simulink model "turbo_controller"  (R2025a)
settings: Solver=FixedStepAuto  StartTime=0.0  StopTime=inf  FixedStep=0.001  RelTol=1e-3
PostLoadFcn:
  | % 自动定位同目录CubeMX文件；不需要外部初始化脚本。
  | codertarget.data.setParameterValue('turbo_controller','STM32CubeMX.ProjectFile',fullfile(fileparts(get_param('turbo_controller','FileName')),'turbo_f407.ioc'));
InitFcn:
  | % 中文说明：按原控制器字段与类型创建三组接口总线；控制参数已内嵌。
  | tc_names=["EValve_Cycle" "EValve_Open" "Eblast_Cycle" "Eblast_Open" "Motor_Cycle" "Motor_Open" "EValve_Enable" "Eblast_Enable" "Motor_Enable" "SWO_Firework" "SWO_BleedAir" "EngineState" "Flag_ECUReset_Clear" "Flag_ECUReset_Save" "Flag_Reset_Enable" "Accelerator" "Nc_dem" "Nc"]; tc_types=["uint16" "uint16" "uint16" "uint16" "uint16" "uint16" "uint8" "uint8" "uint8" "uint8" "uint8" "uint8" "uint8" "uint8" "uint8" "single" "single" "single"];
  | for tc_k=1:numel(tc_names)
  |  tc_e(tc_k)=Simulink.BusElement; tc_e(tc_k).Name=char(tc_names(tc_k)); tc_e(tc_k).DataType=char(tc_types(tc_k));
  | end
  | EngineControl_Out=Simulink.Bus; EngineControl_Out.DataScope='Exported'; EngineControl_Out.Elements=tc_e;
  | clear tc_e tc_names tc_types tc_k
  | tc_names=["savedata1" "savedata2" "savedata3" "savedata4" "savedata5" "savedata6" "savedata7" "savedata8" "savedata9" "savedata10" "savedata11" "savedata12" "savedata13" "savedata14" "savedata15" "savedata16" "savedata17" "savedata18" "savedata19" "savedata20" "savedata21" "savedata22" "savedata23" "savedata24" "savedata25"]; tc_types=["single" "single" "single" "single" "single" "single" "single" "single" "single" "single" "single" "single" "single" "single" "single" "single" "single" "single" "single" "single" "single" "single" "single" "single" "single"];
  | for tc_k=1:numel(tc_names)
  |  tc_e(tc_k)=Simulink.BusElement; tc_e(tc_k).Name=char(tc_names(tc_k)); tc_e(tc_k).DataType=char(tc_types(tc_k));
  | end
  | SaveData_Out=Simulink.Bus; SaveData_Out.DataScope='Exported'; SaveData_Out.Elements=tc_e;
  | clear tc_e tc_names tc_types tc_k
  | tc_names=["senddata1" "senddata2" "senddata3" "senddata4" "senddata5" "senddata6" "senddata7" "senddata8" "senddata9" "senddata10" "senddata11" "senddata12" "senddata13" "senddata14" "senddata15" "senddata16" "senddata17" "senddata18" "senddata19" "senddata20" "senddata21" "senddata22" "senddata23" "senddata24" "senddata25" "senddata26" "senddata27" "senddata28" "senddata29"]; tc_types=["uint8" "uint8" "uint8" "uint8" "uint8" "uint8" "uint8" "uint8" "uint8" "uint8" "uint8" "uint8" "uint8" "uint8" "uint8" "uint8" "uint8" "uint8" "uint8" "uint8" "uint8" "uint8" "uint8" "uint8" "uint8" "uint8" "uint8" "uint8" "uint8"];
  | for tc_k=1:numel(tc_names)
  |  tc_e(tc_k)=Simulink.BusElement; tc_e(tc_k).Name=char(tc_names(tc_k)); tc_e(tc_k).DataType=char(tc_types(tc_k));
  | end
  | SendData_Out=Simulink.Bus; SendData_Out.DataScope='Exported'; SendData_Out.Elements=tc_e;
  | clear tc_e tc_names tc_types tc_k
  | 
  | % 以下为接口中文说明；只设置描述，不改变数值或数据类型。
  | EngineControl_Out.Description='执行控制输出（阀、电机、点火、状态及复位请求）';
  | tc_cn=["EValve_Cycle（主油阀周期计数（每计数2毫秒））" "EValve_Open（主油阀开通计数（每计数2毫秒））" "Eblast_Cycle（副油阀周期计数（每计数2毫秒））" "Eblast_Open（副油阀开通计数（每计数2毫秒））" "Motor_Cycle（起动电机周期计数）" "Motor_Open（起动电机开通计数）" "EValve_Enable（主油阀驱动使能）" "Eblast_Enable（副油阀驱动使能）" "Motor_Enable（起动电机使能）" "SWO_Firework（点火器使能（1开））" "SWO_BleedAir（引气阀使能（1开））" "EngineState（发动机状态）" "Flag_ECUReset_Clear（清除复位恢复状态请求）" "Flag_ECUReset_Save（保存复位恢复数据请求）" "Flag_Reset_Enable（处理器软件复位请求）" "Accelerator（油门／油泵给定控制量）" "Nc_dem（控制目标转速）" "Nc（发动机反馈转速（转每分））"];
  | tc_elements=EngineControl_Out.Elements;
  | for tc_k=1:numel(tc_cn)
  |  tc_elements(tc_k).Description=char(tc_cn(tc_k));
  | end
  | EngineControl_Out.Elements=tc_elements;
  | clear tc_cn tc_elements tc_k
  | SaveData_Out.Description='25项运行记录；字段含义按当前模型数据来源解释';
  | tc_cn=["savedata1（指令回显记录）" "savedata2（入口总温记录（℃））" "savedata3（电源电压记录）" "savedata4（排气温度记录（℃））" "savedata5（标定燃油压力记录）" "savedata6（副油阀占空比记录（％））" "savedata7（主油阀占空比记录（％））" "savedata8（温度修正转速记录）" "savedata9（开关输出及反馈位域）" "savedata10（物理转速记录）" "savedata11（油泵目标给定原始值）" "savedata12（起动电机占空比记录（％））" "savedata13（发动机状态码记录）" "savedata14（故障告警位域记录）" "savedata15（模型记录帧序号）" "savedata16（处理器温度记录（℃））" "savedata17（装订转速记录（沿用旧电源字段名））" "savedata18（导航高度记录）" "savedata19（飞行空速记录）" "savedata20（主阀旧记录位（恒零保留））" "savedata21（第21项保留记录（恒零））" "savedata22（保留记录项22）" "savedata23（保留记录项23）" "savedata24（保留记录项24）" "savedata25（保留记录项25）"];
  | tc_elements=SaveData_Out.Elements;
  | for tc_k=1:numel(tc_cn)
  |  tc_elements(tc_k).Description=char(tc_cn(tc_k));
  | end
  | SaveData_Out.Elements=tc_elements;
  | clear tc_cn tc_elements tc_k
  | SendData_Out.Description='29字段回传及外设命令接口；板端上位机帧只取第3至27字段';
  | tc_cn=["senddata1（回传发送允许标志（不直接上线路））" "senddata2（回传载荷长度25字节）" "senddata3（回传指令回显字节）" "senddata4（总温编码字节（℃＋80））" "senddata5（电源电压编码字节）" "senddata6（排温编码高字节）" "senddata7（排温编码低字节）" "senddata8（燃油压力编码高字节）" "senddata9（燃油压力编码低字节）" "senddata10（副油阀占空比字节（％））" "senddata11（主油阀占空比字节（％））" "senddata12（修正转速编码高字节）" "senddata13（修正转速编码低字节）" "senddata14（驱动及反馈状态位域）" "senddata15（物理转速编码高字节）" "senddata16（物理转速编码低字节）" "senddata17（油泵目标给定高字节（串口二使用））" "senddata18（油泵目标给定低字节（串口二使用））" "senddata19（起动电机占空比命令（串口一使用））" "senddata20（发动机状态码字节）" "senddata21（故障告警位域字节）" "senddata22（帧序号占位（板端另行填写））" "senddata23（处理器温度编码（℃＋50））" "senddata24（控制目标转速编码高字节）" "senddata25（控制目标转速编码低字节）" "senddata26（占位字节（板端改填实测泵速高字节））" "senddata27（占位字节（板端改填实测泵速低字节））" "senddata28（装订转速高字节（本板未发送））" "senddata29（装订转速低字节（本板未发送））"];
  | tc_elements=SendData_Out.Elements;
  | for tc_k=1:numel(tc_cn)
  |  tc_elements(tc_k).Description=char(tc_cn(tc_k));
  | end
  | SendData_Out.Elements=tc_elements;
  | clear tc_cn tc_elements tc_k
  | 
  | 
  | % FRAM模块化事务：接口类型和上电初始状态，随模型保存，无外部初始化文件。
  | clear FM_elements
  | FM_elements(1)=Simulink.BusElement;FM_elements(1).Name='phase';FM_elements(1).DataType='uint8';FM_elements(1).Dimensions=[1 1];FM_elements(1).Description='phase（当前事务阶段）';
  | FM_elements(2)=Simulink.BusElement;FM_elements(2).Name='a';FM_elements(2).DataType='uint8';FM_elements(2).Dimensions=[64 1];FM_elements(2).Description='a（启动时缓存的首区64字节）';
  | FM_elements(3)=Simulink.BusElement;FM_elements(3).Name='active';FM_elements(3).DataType='uint16';FM_elements(3).Dimensions=[1 1];FM_elements(3).Description='active（当前有效记录区地址）';
  | FM_elements(4)=Simulink.BusElement;FM_elements(4).Name='generation';FM_elements(4).DataType='uint32';FM_elements(4).Dimensions=[1 1];FM_elements(4).Description='generation（当前有效记录代号）';
  | FM_elements(5)=Simulink.BusElement;FM_elements(5).Name='record';FM_elements(5).DataType='uint8';FM_elements(5).Dimensions=[64 1];FM_elements(5).Description='record（本次冻结的待写记录）';
  | FM_elements(6)=Simulink.BusElement;FM_elements(6).Name='addr';FM_elements(6).DataType='uint16';FM_elements(6).Dimensions=[1 1];FM_elements(6).Description='addr（本次备用写入地址）';
  | FM_elements(7)=Simulink.BusElement;FM_elements(7).Name='lastSave';FM_elements(7).DataType='single';FM_elements(7).Dimensions=[1 1];FM_elements(7).Description='lastSave（上次开始保存的秒数）';
  | FM_elements(8)=Simulink.BusElement;FM_elements(8).Name='lastState';FM_elements(8).DataType='uint8';FM_elements(8).Dimensions=[1 1];FM_elements(8).Description='lastState（上次保存时的发动机状态）';
  | FM_elements(9)=Simulink.BusElement;FM_elements(9).Name='boot';FM_elements(9).DataType='boolean';FM_elements(9).Dimensions=[1 1];FM_elements(9).Description='boot（启动记录是否允许恢复）';
  | FM_elements(10)=Simulink.BusElement;FM_elements(10).Name='consumed';FM_elements(10).DataType='boolean';FM_elements(10).Dimensions=[1 1];FM_elements(10).Description='consumed（本次启动恢复通知是否已发送）';
  | FM_elements(11)=Simulink.BusElement;FM_elements(11).Name='payload';FM_elements(11).DataType='uint8';FM_elements(11).Dimensions=[20 1];FM_elements(11).Description='payload（当前20字节恢复内容）';
  | ... (+35 lines)
model workspace (MAT data in the model file):
  CRC16_Table_Reference = [0 4129 8258 12387 16516 20645 24774 28903 33032 37161 41290 45419 ... (256 elements, 256x1)]
  PE_Kaer = [0.15402 0.15402 0.12264 0.10076 0.09481 0.07601 0.07111 0.0569 0.05198 0.04926 0.05308 0.04325 ... (13 elements, 1x13)]
  PE_Nr = [21.2982 61.4260372 67.7475458 72.7394382 76.845934 80.6988798 83.8449282 86.6491912 88.9382406 89.178606 91.1938214 93.4068058 ... (13 elements, 1x13)]
  PE_Pump_Translate = 33.5999984741
  PE_RotaSpeed_Translate = 860
  PE_Taer = [0.4939154 0.4939154 0.40780982 0.34066978 0.31622756 0.30405716 0.34300244 0.26785022 0.37393554 0.23914836 0.44563948 0.31044662 ... (13 elements, 1x13)]
  PF_ACCFULLRANGE = 3360
  PF_Flag_ECUReset = 0
  PF_Flag_rx_suc = 1
  PF_Gear_Info = [40000; 45000; 50000; 55000; 57000; 59000; 60000; 61000; 61000; 61000; 61000; 61000]
  PF_K_TiaoJie = 1
  PF_Kpu = 10
  PF_MySet_Rxdata = [0 0 0 0 0 0 0 0 0 0 0 0 ... (50 elements, 50x1)]
  PF_MyUsart1_Rxdata = [0 0 0 0 0 0 0 0 0 0 0 0 ... (50 elements, 50x1)]
  PF_MyUsart2_Rxdata = [0 0 0 0 0 0 0 0 0 0 0 0 ... (50 elements, 50x1)]
  PF_Reset_Information = [0 0 0 0 0 0 0 0 0 0 0 0 ... (20 elements, 20x1)]
  PF_Sensor_X1_T4 = [0 4095]
  PF_Sensor_X2_T4 = [0 1.66666698456]
  PF_Sensor_X3_T4 = [0 504 999 1497 2010 2529 3051 3568 4076 4571 4959]
  PF_Sensor_X_P2 = [0.5 3]
  PF_Sensor_X_Poil = [0.5 3]
  PF_Sensor_X_T1t = [-50 300]
  PF_Sensor_X_Vpower = [0 3]
  PF_Sensor_X_Vpump = [0 3]
  PF_Sensor_Y1_T4 = [0 3]
  PF_Sensor_Y2_T4 = [0 5000]
  PF_Sensor_Y3_T4 = [0 100 200 300 400 500 600 700 800 900 980]
  PF_Sensor_Y_P2 = [0 1000]
  PF_Sensor_Y_Poil = [0 1000]
  PF_Sensor_Y_T1t = [-50 300]
  PF_Sensor_Y_Vpower = [0 33]
  PF_Sensor_Y_Vpump = [0 33]
  PG_CtrlMode_CloseLoop : mpt.Parameter (value not decoded)
  PG_CtrlMode_ManualAcc : mpt.Parameter (value not decoded)
  PG_CtrlMode_Origin : mpt.Parameter (value not decoded)
  PG_CtrlMode_Start : mpt.Parameter (value not decoded)
  PG_CtrlMode_Stop : mpt.Parameter (value not decoded)
  PG_ES_Clp : mpt.Parameter (value not decoded)
  PG_ES_EngStart : mpt.Parameter (value not decoded)
  PG_ES_Manual : mpt.Parameter (value not decoded)
  PG_ES_Origin : mpt.Parameter (value not decoded)
  PG_ES_Stop : mpt.Parameter (value not decoded)
  PG_Instr_BleedAirSet : mpt.Parameter (value not decoded)
  PG_Instr_CloseLoop : mpt.Parameter (value not decoded)
  PG_Instr_ECUReSet : mpt.Parameter (value not decoded)
  PG_Instr_EValveSet : mpt.Parameter (value not decoded)
  PG_Instr_EblastSet : mpt.Parameter (value not decoded)
  PG_Instr_Erase : mpt.Parameter (value not decoded)
  PG_Instr_FireWorkSet : mpt.Parameter (value not decoded)
  PG_Instr_ManualPlus : mpt.Parameter (value not decoded)
  PG_Instr_ManualrReduce : mpt.Parameter (value not decoded)
  PG_Instr_MotorSet : mpt.Parameter (value not decoded)
  PG_Instr_OilSet : mpt.Parameter (value not decoded)
  PG_Instr_SelfCheck : mpt.Parameter (value not decoded)
  PG_Instr_Start : mpt.Parameter (value not decoded)
  PG_Instr_Stop : mpt.Parameter (value not decoded)
  PG_Instr_StopZero : Simulink.Parameter (value not decoded)
  PG_Location_Air : Simulink.Parameter (value not decoded)
  PG_Location_Gnd : Simulink.Parameter (value not decoded)
  PG_ServoCtrlMode_CloseLoop : Simulink.Parameter (value not decoded)
  PG_ServoCtrlMode_CloseLoopMax : Simulink.Parameter (value not decoded)
  PG_ServoCtrlMode_CloseLoopMin : Simulink.Parameter (value not decoded)
  PG_ServoCtrlMode_ManualAcc : Simulink.Parameter (value not decoded)
  PG_ServoCtrlMode_ManualAccMax : Simulink.Parameter (value not decoded)
  PG_ServoCtrlMode_ManualAccMin : Simulink.Parameter (value not decoded)
  PG_SpeedDot_Permit : Simulink.Parameter (value not decoded)
  PL_EngineModel_Actuator = [0 10 100]
  PL_EngineModel_EngineStar_Press_P2 = [1013 1098.4 1099.144828 1099.931034 1103.613793 1162.662069 1143.793103 1131.006897 1123.186207 1117.6 1114 1111.806897 ... (127 elements, 1x127)]
  PL_EngineModel_EngineStar_RotaSpeed = [200 2000 9584 9660 10220 10240 10260 10288 10308 10368 10380 10408 ... (127 elements, 1x127)]
  PL_EngineModel_EngineStar_Temp_Exhaust = [128 129 129.1 130 131 131.1 132 133 134 134.1 135 135.1 ... (127 elements, 1x127)]
  PL_EngineModel_EngineStar_Time = [0.05 0.1 0.15 0.2 0.25 0.3 0.35 0.4 0.45 0.5 0.55 0.6 ... (127 elements, 1x127)]
  PL_EngineModel_IdleAbove_Nr = [0 21.2982 61.4260372 67.7475458 72.7394382 76.845934 80.6988798 83.8449282 86.6491912 88.9382406 89.178606 91.1938214 ... (14 elements, 1x14)]
  PL_EngineModel_IdleAbove_P2r = [0.986923266716 1.57907722675 1.81593881076 1.99358499877 2.23044658278 2.43770046879 2.65482358747 2.84233900814 3.03972366149 3.18776215149 3.25684678016 3.3950160375 ... (14 elements, 1x14)]
  PL_EngineModel_IdleAbove_Tempr = [0.0536001429337 1.07200285867 1.63301768805 1.63659103091 1.66875111667 1.72592460247 1.77595140254 1.86171163123 1.95461854565 2.03323208862 2.03323208862 2.13685903162 ... (14 elements, 1x14)]
  PL_EngineModel_IdleAbove_Ter = [0.42434128 0.42434128 0.42434128 0.30669408 0.23570008 0.22150128 0.1997974 0.23803274 0.16115638 0.24279948 0.13600422 0.31308354 ... (14 elements, 1x14)]
  PL_EngineModel_IdleAbove_Wfr = [0 10.142 23.8337 27.8905 31.9473 36.0041 40.0609 44.1177 48.1745 52.2313 52.7384 56.7952 ... (14 elements, 1x14)]
  PL_EngineModel_Press_P2 = [400 400 400 400 400 400 400 400 400 400]
  PL_EngineModel_Rotaspeed = [0 20000 96400]
  PL_EngineModel_Temp_Exhaust = [500 500 500 500 500 500 500 500 500 500]
  PL_Kaer = [0.1 0.1 0.1 0.1 0.1 0.1]
  PL_Nr = [50 60 70 80 90 100]
  PL_Taer = [0.1 0.1 0.1 0.1 0.1 0.1]
  Sig : Simulink.Signal (value not decoded)
  Ts_ms : Simulink.Parameter (value not decoded)
  false : Simulink.Parameter (value not decoded)
  true : Simulink.Parameter (value not decoded)
symbols that are objects in the model workspace (value not decoded): PG_CtrlMode_CloseLoop, PG_CtrlMode_ManualAcc, PG_CtrlMode_Origin, PG_CtrlMode_Start, PG_CtrlMode_Stop, PG_ES_Clp, PG_ES_EngStart, PG_ES_Manual, PG_ES_Origin, PG_ES_Stop, PG_Instr_BleedAirSet, PG_Instr_CloseLoop, PG_Instr_EblastSet, PG_Instr_ECUReSet, PG_Instr_Erase, PG_Instr_EValveSet, PG_Instr_FireWorkSet, PG_Instr_ManualPlus, PG_Instr_ManualrReduce, PG_Instr_MotorSet, PG_Instr_OilSet, PG_Instr_SelfCheck, PG_Instr_Start, PG_Instr_Stop, PG_Instr_StopZero, PG_ServoCtrlMode_CloseLoop, PG_ServoCtrlMode_CloseLoopMax, PG_ServoCtrlMode_CloseLoopMin, PG_ServoCtrlMode_ManualAcc, PG_ServoCtrlMode_ManualAccMax, PG_ServoCtrlMode_ManualAccMin, Ts_ms
libraries: simulink x97, stm32blockslib x10, stm32f4xxblockslib x8
(part 25 of 26)

== stateflow chart turbo_controller/CLM/Start/Start_OpenLoop ==
  note: 普通起动的六阶段顺序控制
      |
      | A准备：等待约1 s，记录并限制起动前油压参考，设置阀门周期、开启主副油路及电机使能。
      | B拖转：转速达到1000后进入C，开启点火并给出起动供油；约6 s仍未达到要求时走异常退出。
      | C建立油路：经过约3 s、油压相对基准上升50或已有进入标志时，调整主油阀与泵给定；按t、T参数和
      | 转速条件逐渐提高电机开通，达到100进入D。
      | D继续加速：转速超过参数n1进入E；超过约6 s未满足条件时撤销点火、清供油并设置异常阶段码。
      | E按转速供油：泵给定在(n1,m1)、(n2,m2)间按直线计算；超过13000时撤销起动电机和点火，超过2000
      | 0进入F。油压持续高于700或本阶段约30 s超时也有退出分支。
      | F转闭环：转速超过28000或达到约20 s时关闭副油路；再按1 s、3 s的延迟恢复主油路和m4给定，最后
      | 申请进入闭环。
      |
      | 转速单位rpm，T4为温度，油压阈值采用标定后的工程编码。计时统一按毫秒/Ts_ms比较；Ts_ms=20 ms
      | 时，1000 ms对应50次调用。泵曲线公式：
      | 泵给定=m1+(m2-m1)×(当前转速-n1)/(n2-n1)。
      |
      | 这些阶段是流程标志，不是额外的AirStart或BWStart模式。电机关闭还有高转速及锁存路径，最终输
      | 出仍受父级模式和使能控制。
  (default) -> (junction 24)
    settings: description=无附加条件的迁移路径，执行次序1；沿本图当前连接推进。
  (junction 24) -> (junction 458) [order 1] : [Start_A/*起动阶段或中间量编号*/  == true/*真值*/]
    settings: description=本路径的判据/动作：[Start_A == true]。执行次序1；条件成立才执行本箭头动作。
  (junction 458) -> (junction 1346) [order 1] : [CNT_Start_A/*计数器起动阶段或中间量编号*/ >= (1000/Ts_ms/*采样周期毫秒*/)]
    settings: description=本路径的判据/动作：[CNT_Start_A >= (1000/Ts_ms)]。执行次序1；条件成立才执行本箭头动作。
  (junction 1346) -> (junction 1355) [order 1] : [POil/*标定燃油压力*/<50]
    settings: description=本路径的判据/动作：[POil<50]。执行次序1；条件成立才执行本箭头动作。
  (junction 24) -> (junction 463) [order 2]
    settings: description=无附加条件的迁移路径，执行次序2；沿本图当前连接推进。
  (junction 458) -> (junction 466) [order 2] : {Motor_Cycle/*起动电机周期计数*/ = 100;
      | Motor_Open/*起动电机开通计数*/ = NPump0/*油泵转速0*/;
      | Motor_Enable/*起动电机使能*/ = uint8/*八位无符号整数*/(1);
      | Eblast_Cycle/*副油阀周期计数（每计数2毫秒）*/ = 30;
      | Eblast_Open/*副油阀开通计数（每计数2毫秒）*/ = 30;
      | Eblast_Enable/*副油阀驱动使能*/ = uint8/*八位无符号整数*/(1);
      | EValve_Cycle/*主油阀周期计数（每计数2毫秒）*/ = 30;
      | EValve_Open/*主油阀开通计数（每计数2毫秒）*/ = 30;
      | EValve_Enable/*主油阀驱动使能*/ = uint8/*八位无符号整数*/(1);}
    settings: description=本路径的判据/动作：{Motor_Cycle = 100; Motor_Open = NPump0; Motor_Enable = uint8(1); Eblast_Cycle = 30; Eblast_Open = 30; Eblast_Enable = uint8(1); EValve_Cycle = 30; EValve_Open = 30; EValve_Enable = uint8(1);}。执行次序2；条件成立才执行本箭头动作。
  (junction 1346) -> (junction 1359) [order 2]
    settings: description=无附加条件的迁移路径，执行次序2；沿本图当前连接推进。
  (junction 1355) -> (junction 1357) : {Origin_POil_m/*原位油压中位或中间变量*/=50;}
    settings: description=本路径的判据/动作：{Origin_POil_m=50;}。执行次序1；条件成立才执行本箭头动作。
  (junction 1359) -> (junction 1361) [order 1] : [POil/*标定燃油压力*/>100]
    settings: description=本路径的判据/动作：[POil>100]。执行次序1；条件成立才执行本箭头动作。
  (junction 1359) -> (junction 1365) [order 2] : {Origin_POil_m/*原位油压中位或中间变量*/=POil/*标定燃油压力*/;}
    settings: description=本路径的判据/动作：{Origin_POil_m=POil;}。执行次序2；条件成立才执行本箭头动作。
  (junction 1361) -> (junction 1363) : {Origin_POil_m/*原位油压中位或中间变量*/=100;}
    settings: description=本路径的判据/动作：{Origin_POil_m=100;}。执行次序1；条件成立才执行本箭头动作。
  (junction 1363) -> (junction 1365)
    settings: description=无附加条件的迁移路径，执行次序1；沿本图当前连接推进。
  (junction 1357) -> (junction 1363)
    settings: description=无附加条件的迁移路径，执行次序1；沿本图当前连接推进。
  (junction 1365) -> (junction 1348) : {Start_A/*起动阶段或中间量编号*/ = false/*假值*/;
      | Start_B/*起动阶段或中间量编号*/ = true/*真值*/;}
    settings: description=本路径的判据/动作：{Start_A = false; Start_B = true;}。执行次序1；条件成立才执行本箭头动作。
  (junction 466) -> (junction 463) : {CNT_Start_A/*计数器起动阶段或中间量编号*/++;}
    settings: description=本路径的判据/动作：{CNT_Start_A++;}。执行次序1；条件成立才执行本箭头动作。
  (junction 1348) -> (junction 466)
    settings: description=无附加条件的迁移路径，执行次序1；沿本图当前连接推进。
  (junction 463) -> (junction 209)
    settings: description=无附加条件的迁移路径，执行次序1；沿本图当前连接推进。
  (junction 209) -> (junction 460) [order 1] : [Start_B/*起动阶段或中间量编号*/  == true/*真值*/]
    settings: description=本路径的判据/动作：[Start_B == true]。执行次序1；条件成立才执行本箭头动作。
  (junction 460) -> (junction 474) [order 1] : [Nc/*发动机反馈转速（转每分）*/ >= 1000 ]
    settings: description=本路径的判据/动作：[Nc >= 1000 ]。执行次序1；条件成立才执行本箭头动作。
  (junction 209) -> (junction 472) [order 2]
    settings: description=无附加条件的迁移路径，执行次序2；沿本图当前连接推进。
  (junction 460) -> (junction 1003) [order 2]
    settings: description=无附加条件的迁移路径，执行次序2；沿本图当前连接推进。
  (junction 474) -> (junction 479) : {Start_B/*起动阶段或中间量编号*/ = false/*假值*/;
      | Start_C/*起动条件输入或阶段编号*/ = true/*真值*/;
      | SWO_Firework/*点火器使能（1开）*/ = uint8/*八位无符号整数*/(1);
      | Accelerator/*油门／油泵给定控制量*/ = 5000;
      | T4_01/*原工程排气温度01*/=T4/*排气温度（℃）*/;}
    settings: description=本路径的判据/动作：{Start_B = false; Start_C = true; SWO_Firework = uint8(1); Accelerator = 5000; T4_01=T4;}。执行次序1；条件成立才执行本箭头动作。
  (junction 1003) -> (junction 998) [order 1] : [CNT_Start_B/*计数器起动阶段或中间量编号*/ >= (6000/Ts_ms/*采样周期毫秒*/)]
    settings: description=本路径的判据/动作：[CNT_Start_B >= (6000/Ts_ms)]。执行次序1；条件成立才执行本箭头动作。
  (junction 1003) -> (junction 476) [order 2]
    settings: description=无附加条件的迁移路径，执行次序2；沿本图当前连接推进。
  (junction 998) -> (junction 1001) : {Flag_EngineState/*标志发动机状态*/= 4;
      | Motor_Open/*起动电机开通计数*/ = 0;}
    settings: description=本路径的判据/动作：{Flag_EngineState= 4; Motor_Open = 0;}。执行次序1；条件成立才执行本箭头动作。
  (junction 476) -> (junction 472) : {CNT_Start_B/*计数器起动阶段或中间量编号*/++;}
    settings: description=本路径的判据/动作：{CNT_Start_B++;}。执行次序1；条件成立才执行本箭头动作。
  (junction 1001) -> (junction 476)
    settings: description=无附加条件的迁移路径，执行次序1；沿本图当前连接推进。
  (junction 479) -> (junction 1001)
    settings: description=无附加条件的迁移路径，执行次序1；沿本图当前连接推进。
  (junction 472) -> (junction 492)
    settings: description=无附加条件的迁移路径，执行次序1；沿本图当前连接推进。
  (junction 492) -> (junction 1307) [order 1] : [Start_C/*起动条件输入或阶段编号*/  == true/*真值*/]
    settings: description=本路径的判据/动作：[Start_C == true]。执行次序1；条件成立才执行本箭头动作。
  (junction 1307) -> (junction 1156) [order 1] : [(((CNT_Start_C/*计数器起动条件输入或阶段编号*/) > (3000/Ts_ms/*采样周期毫秒*/))  ||  (POil/*标定燃油压力*/-Origin_POil/*原位油压*/>=50))||Flag_IntoC/*标志进入条件输入或阶段编号*/]
    settings: description=本路径的判据/动作：[(((CNT_Start_C) > (3000/Ts_ms)) || (POil-Origin_POil>=50))||Flag_IntoC]。执行次序1；条件成立才执行本箭头动作。
  (junction 492) -> (junction 577) [order 2]
    settings: description=无附加条件的迁移路径，执行次序2；沿本图当前连接推进。
  (junction 1307) -> (junction 1334) [order 2]
    settings: description=无附加条件的迁移路径，执行次序2；沿本图当前连接推进。
  (junction 1156) -> (junction 1337) : {EValve_Cycle/*主油阀周期计数（每计数2毫秒）*/ = 30;
      | EValve_Open/*主油阀开通计数（每计数2毫秒）*/ = 0;
      | EValve_Enable/*主油阀驱动使能*/ = uint8/*八位无符号整数*/(0);
      | Accelerator/*油门／油泵给定控制量*/ = m1/*中位或中间变量1*/;}
    settings: description=本路径的判据/动作：{EValve_Cycle = 30; EValve_Open = 0; EValve_Enable = uint8(0); Accelerator = m1;}。执行次序1；条件成立才执行本箭头动作。
  (junction 1334) -> (junction 1158)
    settings: description=无附加条件的迁移路径，执行次序1；沿本图当前连接推进。
  (junction 1337) -> (junction 494) [order 1] : [((CNT_Start_C1/*计数器起动条件输入或阶段编号1*/) >=(t/*温度、时间或真分支输入*/*1000/Ts_ms/*采样周期毫秒*/)  ||  ( Nc/*发动机反馈转速（转每分）*/>=6000 ))||Flag_IntoC/*标志进入条件输入或阶段编号*/]
    settings: description=本路径的判据/动作：[((CNT_Start_C1) >=(t*1000/Ts_ms) || ( Nc>=6000 ))||Flag_IntoC]。执行次序1；条件成立才执行本箭头动作。
  (junction 494) -> (junction 1374)
    settings: description=无附加条件的迁移路径，执行次序1；沿本图当前连接推进。
  (junction 1374) -> (junction 1380) [order 1] : [Motor_Open/*起动电机开通计数*/>=100]
    settings: description=本路径的判据/动作：[Motor_Open>=100]。执行次序1；条件成立才执行本箭头动作。
  (junction 1337) -> (junction 1178) [order 2] : {CNT_Start_C1/*计数器起动条件输入或阶段编号1*/++;}
    settings: description=本路径的判据/动作：{CNT_Start_C1++;}。执行次序2；条件成立才执行本箭头动作。
  (junction 1374) -> (junction 1375) [order 2] : {Motor_Open/*起动电机开通计数*/ = Motor_Open/*起动电机开通计数*/+(100-NPump0/*油泵转速0*/)/(T/*温度、时间或真分支输入*/*1000/Ts_ms/*采样周期毫秒*/);
      | Flag_IntoC/*标志进入条件输入或阶段编号*/=true/*真值*/;}
    settings: description=本路径的判据/动作：{Motor_Open = Motor_Open+(100-NPump0)/(T*1000/Ts_ms); Flag_IntoC=true;}。执行次序2；条件成立才执行本箭头动作。
  (junction 1380) -> (junction 1381) : {Start_C/*起动条件输入或阶段编号*/ = false/*假值*/;
      | Start_D/*起动阶段或中间量编号*/= true/*真值*/;
      | Motor_Open/*起动电机开通计数*/ = 100;}
    settings: description=本路径的判据/动作：{Start_C = false; Start_D= true; Motor_Open = 100;}。执行次序1；条件成立才执行本箭头动作。
  (junction 1158) -> (junction 577) : {CNT_Start_C/*计数器起动条件输入或阶段编号*/++;}
    settings: description=本路径的判据/动作：{CNT_Start_C++;}。执行次序1；条件成立才执行本箭头动作。
  (junction 1178) -> (junction 1158)
    settings: description=无附加条件的迁移路径，执行次序1；沿本图当前连接推进。
  (junction 1339) -> (junction 1178)
    settings: description=无附加条件的迁移路径，执行次序1；沿本图当前连接推进。
  (junction 1191) -> (junction 1339)
    settings: description=无附加条件的迁移路径，执行次序1；沿本图当前连接推进。
  (junction 1375) -> (junction 1191)
    settings: description=无附加条件的迁移路径，执行次序1；沿本图当前连接推进。
  (junction 1381) -> (junction 1375)
    settings: description=无附加条件的迁移路径，执行次序1；沿本图当前连接推进。
  (junction 577) -> (junction 585)
    settings: description=无附加条件的迁移路径，执行次序1；沿本图当前连接推进。
  (junction 585) -> (junction 592) [order 1] : [Start_D/*起动阶段或中间量编号*/ == true/*真值*/]
    settings: description=本路径的判据/动作：[Start_D == true]。执行次序1；条件成立才执行本箭头动作。
  (junction 592) -> (junction 801) [order 1] : [Nc/*发动机反馈转速（转每分）*/>n1/*转速变量1*/]
    settings: description=本路径的判据/动作：[Nc>n1]。执行次序1；条件成立才执行本箭头动作。
  (junction 592) -> (junction 1192) [order 2]
    settings: description=无附加条件的迁移路径，执行次序2；沿本图当前连接推进。
  (junction 585) -> (junction 594) [order 2]
    settings: description=无附加条件的迁移路径，执行次序2；沿本图当前连接推进。
  (junction 801) -> (junction 803) : {Start_D/*起动阶段或中间量编号*/ = false/*假值*/;
      | Start_E/*起动阶段或中间量编号*/ = true/*真值*/;}
    settings: description=本路径的判据/动作：{Start_D = false; Start_E = true;}。执行次序1；条件成立才执行本箭头动作。
  (junction 1192) -> (junction 1166)
    settings: description=无附加条件的迁移路径，执行次序1；沿本图当前连接推进。
  (junction 1166) -> (junction 1170) [order 1] : [(CNT_Start_D/*计数器起动阶段或中间量编号*/) > (6000/Ts_ms/*采样周期毫秒*/)]
    settings: description=本路径的判据/动作：[(CNT_Start_D) > (6000/Ts_ms)]。执行次序1；条件成立才执行本箭头动作。
  (junction 1166) -> (junction 910) [order 2]
    settings: description=无附加条件的迁移路径，执行次序2；沿本图当前连接推进。
  (junction 1170) -> (junction 1168) : {SWO_Firework/*点火器使能（1开）*/ = uint8/*八位无符号整数*/(0);
      | Flag_EngineState/*标志发动机状态*/= 15;
      | Accelerator/*油门／油泵给定控制量*/ =0;}
    settings: description=本路径的判据/动作：{SWO_Firework = uint8(0); Flag_EngineState= 15; Accelerator =0;}。执行次序1；条件成立才执行本箭头动作。
  (junction 1168) -> (junction 910)
    settings: description=无附加条件的迁移路径，执行次序1；沿本图当前连接推进。
  (junction 1194) -> (junction 1168)
    settings: description=无附加条件的迁移路径，执行次序1；沿本图当前连接推进。
  (junction 803) -> (junction 1194)
    settings: description=无附加条件的迁移路径，执行次序1；沿本图当前连接推进。
  (junction 910) -> (junction 594) : {CNT_Start_D/*计数器起动阶段或中间量编号*/++;}
    settings: description=本路径的判据/动作：{CNT_Start_D++;}。执行次序1；条件成立才执行本箭头动作。
  (junction 594) -> (junction 621)
    settings: description=无附加条件的迁移路径，执行次序1；沿本图当前连接推进。
  (junction 621) -> (junction 1202) [order 1] : [Start_E/*起动阶段或中间量编号*/ == true/*真值*/]
    settings: description=本路径的判据/动作：[Start_E == true]。执行次序1；条件成立才执行本箭头动作。
  (junction 1202) -> (junction 1249) [order 1] : [(Nc/*发动机反馈转速（转每分）*/ > 20000) ]
    settings: description=本路径的判据/动作：[(Nc > 20000) ]。执行次序1；条件成立才执行本箭头动作。
  (junction 621) -> (junction 357) [order 2]
    settings: description=无附加条件的迁移路径，执行次序2；沿本图当前连接推进。
  (junction 1202) -> (junction 1231) [order 2]
    settings: description=无附加条件的迁移路径，执行次序2；沿本图当前连接推进。
  (junction 1249) -> (junction 1251) : {Start_E/*起动阶段或中间量编号*/ = false/*假值*/;
      | Start_F/*起动假分支输入或函数变量*/= true/*真值*/;
      | Motor_Cycle/*起动电机周期计数*/ = 100;
      | Motor_Open/*起动电机开通计数*/ = 0;
      | Motor_Enable/*起动电机使能*/ = uint8/*八位无符号整数*/(0);
      | SWO_Firework/*点火器使能（1开）*/ = uint8/*八位无符号整数*/(0);
      | Accelerator/*油门／油泵给定控制量*/ =m3/*中位或中间变量3*/;}
    settings: description=本路径的判据/动作：{Start_E = false; Start_F= true; Motor_Cycle = 100; Motor_Open = 0; Motor_Enable = uint8(0); SWO_Firework = uint8(0); Accelerator =m3;}。执行次序1；条件成立才执行本箭头动作。
  (junction 1231) -> (junction 1226) [order 1] : [POil/*标定燃油压力*/>700]
    settings: description=本路径的判据/动作：[POil>700]。执行次序1；条件成立才执行本箭头动作。
  (junction 1231) -> (junction 1255) [order 2]
    settings: description=无附加条件的迁移路径，执行次序2；沿本图当前连接推进。
  (junction 1226) -> (junction 1237)
    settings: description=无附加条件的迁移路径，执行次序1；沿本图当前连接推进。
  (junction 1255) -> (junction 1259) [order 1] : [CNT_Start_E/*计数器起动阶段或中间量编号*/>30000/Ts_ms/*采样周期毫秒*/]
    settings: description=本路径的判据/动作：[CNT_Start_E>30000/Ts_ms]。执行次序1；条件成立才执行本箭头动作。
  (junction 1255) -> (junction 1316) [order 2]
    settings: description=无附加条件的迁移路径，执行次序2；沿本图当前连接推进。
  (junction 1259) -> (junction 1257) : {Flag_EngineState/*标志发动机状态*/= 15;
      | Accelerator/*油门／油泵给定控制量*/ =0;}
    settings: description=本路径的判据/动作：{Flag_EngineState= 15; Accelerator =0;}。执行次序1；条件成立才执行本箭头动作。
  (junction 1316) -> (junction 1318) [order 1] : [Nc/*发动机反馈转速（转每分）*/ > 13000 ]
    settings: description=本路径的判据/动作：[Nc > 13000 ]。执行次序1；条件成立才执行本箭头动作。
  (junction 1316) -> (junction 1323) [order 2]
    settings: description=无附加条件的迁移路径，执行次序2；沿本图当前连接推进。
  (junction 1318) -> (junction 1390) : {Motor_Cycle/*起动电机周期计数*/ = 100;
      | Motor_Open/*起动电机开通计数*/ = 0;
      | Motor_Enable/*起动电机使能*/ = uint8/*八位无符号整数*/(0);
      | SWO_Firework/*点火器使能（1开）*/ = uint8/*八位无符号整数*/(0);}
    settings: description=本路径的判据/动作：{Motor_Cycle = 100; Motor_Open = 0; Motor_Enable = uint8(0); SWO_Firework = uint8(0);}。执行次序1；条件成立才执行本箭头动作。
  (junction 1390) -> (junction 1323)
    settings: description=无附加条件的迁移路径，执行次序1；沿本图当前连接推进。
  (junction 1323) -> (junction 1207) : {Accelerator/*油门／油泵给定控制量*/=(m2/*中位或中间变量2*/-m1/*中位或中间变量1*/)/(n2/*转速变量2*/-n1/*转速变量1*/)*Nc/*发动机反馈转速（转每分）*/+(m1/*中位或中间变量1*/*n2/*转速变量2*/-m2/*中位或中间变量2*/*n1/*转速变量1*/)/(n2/*转速变量2*/-n1/*转速变量1*/);}
    settings: description=本路径的判据/动作：{Accelerator=(m2-m1)/(n2-n1)*Nc+(m1*n2-m2*n1)/(n2-n1);}。执行次序1；条件成立才执行本箭头动作。
  (junction 1237) -> (junction 1239) [order 1] : [CNT_POilHigh/*计数器压力或比例变量油高值*/ > (2000/Ts_ms/*采样周期毫秒*/)]
    settings: description=本路径的判据/动作：[CNT_POilHigh > (2000/Ts_ms)]。执行次序1；条件成立才执行本箭头动作。
  (junction 1237) -> (junction 1228) [order 2] : {CNT_POilHigh/*计数器压力或比例变量油高值*/++;}
    settings: description=本路径的判据/动作：{CNT_POilHigh++;}。执行次序2；条件成立才执行本箭头动作。
  (junction 1239) -> (junction 1240) : {Flag_EngineState/*标志发动机状态*/= 15;
      | Accelerator/*油门／油泵给定控制量*/ =0;}
    settings: description=本路径的判据/动作：{Flag_EngineState= 15; Accelerator =0;}。执行次序1；条件成立才执行本箭头动作。
  (junction 1207) -> (junction 357) : {CNT_Start_E/*计数器起动阶段或中间量编号*/++;}
    settings: description=本路径的判据/动作：{CNT_Start_E++;}。执行次序1；条件成立才执行本箭头动作。
  (junction 1205) -> (junction 1207)
    settings: description=无附加条件的迁移路径，执行次序1；沿本图当前连接推进。
  (junction 1319) -> (junction 1205)
    settings: description=无附加条件的迁移路径，执行次序1；沿本图当前连接推进。
  (junction 1257) -> (junction 1319)
    settings: description=无附加条件的迁移路径，执行次序1；沿本图当前连接推进。
  (junction 1228) -> (junction 1257)
    settings: description=无附加条件的迁移路径，执行次序1；沿本图当前连接推进。
  (junction 1240) -> (junction 1228)
    settings: description=无附加条件的迁移路径，执行次序1；沿本图当前连接推进。
  (junction 1251) -> (junction 1240)
    settings: description=无附加条件的迁移路径，执行次序1；沿本图当前连接推进。
  (junction 357) -> (junction 1135)
    settings: description=无附加条件的迁移路径，执行次序1；沿本图当前连接推进。
  (junction 1135) -> (junction 1268) [order 1] : [Start_F/*起动假分支输入或函数变量*/ == true/*真值*/]
    settings: description=本路径的判据/动作：[Start_F == true]。执行次序1；条件成立才执行本箭头动作。
  (junction 1268) -> (junction 1233) [order 1] : [Nc/*发动机反馈转速（转每分）*/ > 28000 || (CNT_Start_F/*计数器起动假分支输入或函数变量*/>=20000/Ts_ms/*采样周期毫秒*/) ]
    settings: description=本路径的判据/动作：[Nc > 28000 || (CNT_Start_F>=20000/Ts_ms) ]。执行次序1；条件成立才执行本箭头动作。
  (junction 1268) -> (junction 1281) [order 2]
    settings: description=无附加条件的迁移路径，执行次序2；沿本图当前连接推进。
  (junction 1135) -> (junction 1264) [order 2]
    settings: description=无附加条件的迁移路径，执行次序2；沿本图当前连接推进。
  (junction 1233) -> (junction 1299) : {Eblast_Cycle/*副油阀周期计数（每计数2毫秒）*/ = 30;
      | Eblast_Open/*副油阀开通计数（每计数2毫秒）*/ = 0;
      | Eblast_Enable/*副油阀驱动使能*/ = uint8/*八位无符号整数*/(0);}
    settings: description=本路径的判据/动作：{Eblast_Cycle = 30; Eblast_Open = 0; Eblast_Enable = uint8(0);}。执行次序1；条件成立才执行本箭头动作。
  (junction 1281) -> (junction 1287)
    settings: description=无附加条件的迁移路径，执行次序1；沿本图当前连接推进。
  (junction 1299) -> (junction 1298) [order 1] : [CNT_EValve_Open/*计数器主油电磁阀开通计数*/ > (3000/Ts_ms/*采样周期毫秒*/)]
    settings: description=本路径的判据/动作：[CNT_EValve_Open > (3000/Ts_ms)]。执行次序1；条件成立才执行本箭头动作。
  (junction 1299) -> (junction 1296) [order 2]
    settings: description=无附加条件的迁移路径，执行次序2；沿本图当前连接推进。
  (junction 1298) -> (junction 1302) : {Flag_EngineState/*标志发动机状态*/= 2;}
    settings: description=本路径的判据/动作：{Flag_EngineState= 2;}。执行次序1；条件成立才执行本箭头动作。
  (junction 1287) -> (junction 1282)
    settings: description=无附加条件的迁移路径，执行次序1；沿本图当前连接推进。
  (junction 1296) -> (junction 1295) [order 1] : [CNT_EValve_Open/*计数器主油电磁阀开通计数*/ > (1000/Ts_ms/*采样周期毫秒*/)]
    settings: description=本路径的判据/动作：[CNT_EValve_Open > (1000/Ts_ms)]。执行次序1；条件成立才执行本箭头动作。
  (junction 1296) -> (junction 1288) [order 2]
    settings: description=无附加条件的迁移路径，执行次序2；沿本图当前连接推进。
  (junction 1295) -> (junction 1294) : {EValve_Cycle/*主油阀周期计数（每计数2毫秒）*/ = 30;
      | EValve_Open/*主油阀开通计数（每计数2毫秒）*/ = 30;
      | EValve_Enable/*主油阀驱动使能*/ = uint8/*八位无符号整数*/(1);
      | Accelerator/*油门／油泵给定控制量*/ =m4/*中位或中间变量4*/;}
    settings: description=本路径的判据/动作：{EValve_Cycle = 30; EValve_Open = 30; EValve_Enable = uint8(1); Accelerator =m4;}。执行次序1；条件成立才执行本箭头动作。
  (junction 1282) -> (junction 1264) : {CNT_Start_F/*计数器起动假分支输入或函数变量*/++;}
    settings: description=本路径的判据/动作：{CNT_Start_F++;}。执行次序1；条件成立才执行本箭头动作。
  (junction 1285) -> (junction 1282)
    settings: description=无附加条件的迁移路径，执行次序1；沿本图当前连接推进。
  (junction 1283) -> (junction 1285)
    settings: description=无附加条件的迁移路径，执行次序1；沿本图当前连接推进。
  (junction 1288) -> (junction 1283) : {CNT_EValve_Open/*计数器主油电磁阀开通计数*/++;}
    settings: description=本路径的判据/动作：{CNT_EValve_Open++;}。执行次序1；条件成立才执行本箭头动作。
  (junction 1294) -> (junction 1288)
    settings: description=无附加条件的迁移路径，执行次序1；沿本图当前连接推进。
  (junction 1302) -> (junction 1294)
    settings: description=无附加条件的迁移路径，执行次序1；沿本图当前连接推进。
  (junction 1264) -> (junction 1398)
    settings: description=无附加条件的迁移路径，执行次序1；沿本图当前连接推进。
  (junction 1398) -> (junction 1392) [order 1] : [(Nc/*发动机反馈转速（转每分）*/ > 13000)||(Motor_OFF_Enable/*电机关闭使能*/==1) ]
    settings: description=本路径的判据/动作：[(Nc > 13000)||(Motor_OFF_Enable==1) ]。执行次序1；条件成立才执行本箭头动作。
  (junction 1392) -> (junction 1393) [order 1] : [CNT_Motor/*计数器电机*/ > 4]
    settings: description=本路径的判据/动作：[CNT_Motor > 4]。执行次序1；条件成立才执行本箭头动作。
  (junction 1398) -> (junction 1394) [order 2]
    settings: description=无附加条件的迁移路径，执行次序2；沿本图当前连接推进。
  (junction 1392) -> (junction 1395) [order 2] : {CNT_Motor/*计数器电机*/++;}
    settings: description=本路径的判据/动作：{CNT_Motor++;}。执行次序2；条件成立才执行本箭头动作。
  (junction 1393) -> (junction 1396) : {Motor_Cycle/*起动电机周期计数*/ = 100;
      | Motor_Open/*起动电机开通计数*/ = 0;
      | Motor_OFF_Enable/*电机关闭使能*/ = uint8/*八位无符号整数*/(1);
      | }
    settings: description=本路径的判据/动作：{Motor_Cycle = 100; Motor_Open = 0; Motor_OFF_Enable = uint8(1); }。执行次序1；条件成立才执行本箭头动作。
  (junction 1395) -> (junction 1394)
    settings: description=无附加条件的迁移路径，执行次序1；沿本图当前连接推进。
  (junction 1396) -> (junction 1395)
    settings: description=无附加条件的迁移路径，执行次序1；沿本图当前连接推进。
  (junction 1394) -> (junction 1397)
    settings: description=无附加条件的迁移路径，执行次序1；沿本图当前连接推进。
  data: Accelerator output single =0; T4 input single; Nc input single; POil input single; CNT_Start_C local uint32 =0; EValve_Cycle output uint16 =0; EValve_Open output uint16 =0; Eblast_Cycle output uint16 =0; Eblast_Open output uint16 =0; Motor_Cycle output uint16 =0; CNT_Start_E local uint32 =0; CNT_Start_B local uint32 =0; Motor_Open output single =0; EValve_Enable output uint8 =0; Eblast_Enable output uint8 =0; Motor_Enable output uint8 =0; SWO_Firework output uint8 =0; NPump0 input uint16; m1 input single; m2 input single; m3 input single; m4 input single; n1 input single; n2 input single; T input single; t input single; Flag_EngineState output uint8 =0; CNT_Start_F local uint32 =0; Start_A local boolean =1; Start_B local boolean =0; Start_C local boolean =0; Start_D local boolean =0; Start_E local boolean =0; Start_F local boolean =0; Ts_ms input single; CNT_Motor local uint32 =0; CNT_Start_D local uint32 =0; CNT_EValve_Open local uint32 =0; CNT_Start_A local uint32 =0; Origin_POil input single; CNT_POilHigh local uint32 =0; T4_01 local single; CNT_Start_C1 local uint32 =0; Origin_POil_m local single; Flag_IntoC local boolean =0; Motor_OFF_Enable local uint8 =0

== stateflow chart turbo_controller/COMMRead_ISM/CMMRead/T1t_P1t_Cal/H0_T0_计算 ==
  note: 保持环境设定，并按更新条件刷新高度信息
      |
      | sheding条件满足时，把输入H0保存到Load_H，把输入T0保存到T0_out；gaodubianhua条件满足时，把H
      | 0保存到H_GPRS。条件不满足时不重新赋值，输出继续保留上次结果。
      |
      | 当前父级把这两个条件都接到接收更新相关信号，因此更新时机取决于通信帧。两个高度输出虽然都取
      | 自H0，供下游使用的用途不同；不能把它们的名称理解为本图重新计算了两套GPS位置。
      |
      | 本处不执行大气公式，温度转K、高度转km以及总温总压计算在外层完成。
  (default) -> (junction 11)
    settings: description=无附加条件的迁移路径，执行次序1；沿本图当前连接推进。
  (junction 11) -> (junction 12) [order 1] : [sheding == true ... % 设定 == 真
      | ]
    settings: description=本路径的判据/动作：[sheding == true ... % 设定 == 真 ]。执行次序1；条件成立才执行本箭头动作。
  (junction 11) -> (junction 16) [order 2]
    settings: description=无附加条件的迁移路径，执行次序2；沿本图当前连接推进。
  (junction 12) -> (junction 14) : {Load_H = H0;
      | T0_out = T0; % 负载或装订值高字节 = 初始高度;；环境温度输出 = 环境温度;
      | }
    settings: description=本路径的判据/动作：{Load_H = H0; T0_out = T0; % 负载或装订值高字节 = 初始高度;；环境温度输出 = 环境温度; }。执行次序1；条件成立才执行本箭头动作。
  (junction 14) -> (junction 16)
    settings: description=无附加条件的迁移路径，执行次序1；沿本图当前连接推进。
  (junction 16) -> (junction 27)
    settings: description=无附加条件的迁移路径，执行次序1；沿本图当前连接推进。
  (junction 27) -> (junction 23) [order 1] : [gaodubianhua == true ... % 高度变化 == 真
      | ]
    settings: description=本路径的判据/动作：[gaodubianhua == true ... % 高度变化 == 真 ]。执行次序1；条件成立才执行本箭头动作。
  (junction 27) -> (junction 20) [order 2]
    settings: description=无附加条件的迁移路径，执行次序2；沿本图当前连接推进。
  (junction 23) -> (junction 22) : {H_GPRS = H0; % 高字节高度信息通道标识 = 初始高度;
      | }
    settings: description=本路径的判据/动作：{H_GPRS = H0; % 高字节高度信息通道标识 = 初始高度; }。执行次序1；条件成立才执行本箭头动作。
  (junction 22) -> (junction 20)
    settings: description=无附加条件的迁移路径，执行次序1；沿本图当前连接推进。
  (junction 20) -> (junction 30)
    settings: description=无附加条件的迁移路径，执行次序1；沿本图当前连接推进。
  data: sheding input boolean; gaodubianhua input boolean; H0 input single; T0 input single; Load_H output single =single(0); H_GPRS output single =single(0); T0_out output single =single(0)

== stateflow chart turbo_controller/COMMRead_ISM/ISM/AnalogFilter_Nc/GeneralFilter/Xlim_Xdot_Judge ==
  note: 区分转速越界与突然跳变，并控制恢复
      |
      | 先检查当前值是否在X_llim～X_ulim内，再检查与上一拍原始值的变化。幅值超限和变化超限分别产生
      | X_Flag_Locking与Xdot_Flag_Locking。
      |
      | 不接受本拍样本时，输出X_pre，即上一有效输出；接受时输出当前X。这样偶发突跳不会直接冲进闭环
      | 。变化恢复采用更小的Xdot_CancelLim门限，并累计CNT_Xdot，只有超过Xdot_Cancelcycle才解除相应
      | 保持。
      |
      | 门限由父级给定：转速变化检查使用1200，恢复门限800，确认时间100 ms换算为调用次数。比较的是
      | 相邻采样差值，不是已经除以采样周期的rpm/s，不能把1200直接标成加速度单位。
  (default) -> (junction 232)
    settings: description=无附加条件的迁移路径，执行次序1；沿本图当前连接推进。
  (junction 232) -> (junction 234) [order 1] : [(X/*自变量或输入量*/ > X_ulim/*输入上限*/) || (X/*自变量或输入量*/  <  X_llim/*输入下限*/)]
    settings: description=本路径的判据/动作：[(X > X_ulim) || (X < X_llim)]。执行次序1；条件成立才执行本箭头动作。
  (junction 232) -> (junction 33) [order 2]
    settings: description=无附加条件的迁移路径，执行次序2；沿本图当前连接推进。
  (junction 234) -> (junction 240) : {X_Out/*自变量或输入量输出*/ = X_pre/*自变量或输入量前一周期*/;X_Flag_Locking/*自变量或输入量标志锁存*/ = FlagTrue/*真值*/;Xdot_Flag_Locking/*输入变化量标志锁存*/ = FlagFalse/*假值*/;CNT_X/*计数器自变量或输入量*/ = 0;}
    settings: description=本路径的判据/动作：{X_Out = X_pre;X_Flag_Locking = FlagTrue;Xdot_Flag_Locking = FlagFalse;CNT_X = 0;}。执行次序1；条件成立才执行本箭头动作。
  (junction 33) -> (junction 146) [order 1] : [(X_Flag_Locking/*自变量或输入量标志锁存*/ == FlagTrue/*真值*/) && (X/*自变量或输入量*/<= X_ulim/*输入上限*/) && (X/*自变量或输入量*/  >=  X_llim/*输入下限*/)]
    settings: description=本路径的判据/动作：[(X_Flag_Locking == FlagTrue) && (X<= X_ulim) && (X >= X_llim)]。执行次序1；条件成立才执行本箭头动作。
  (junction 33) -> (junction 8) [order 2]
    settings: description=无附加条件的迁移路径，执行次序2；沿本图当前连接推进。
  (junction 146) -> (junction 216) : {CNT_X/*计数器自变量或输入量*/++;}
    settings: description=本路径的判据/动作：{CNT_X++;}。执行次序1；条件成立才执行本箭头动作。
  (junction 8) -> (junction 91) [order 1] : [((X/*自变量或输入量*/-Xin_pre/*输入量前一周期*/) > Xdot_lim/*变化量限值*/) || ((X/*自变量或输入量*/-Xin_pre/*输入量前一周期*/) < -Xdot_lim/*变化量限值*/)]
    settings: description=本路径的判据/动作：[((X-Xin_pre) > Xdot_lim) || ((X-Xin_pre) < -Xdot_lim)]。执行次序1；条件成立才执行本箭头动作。
  (junction 8) -> (junction 190) [order 2]
    settings: description=无附加条件的迁移路径，执行次序2；沿本图当前连接推进。
  (junction 91) -> (junction 187) : {X_Out/*自变量或输入量输出*/ = X_pre/*自变量或输入量前一周期*/;X_Flag_Locking/*自变量或输入量标志锁存*/ = FlagFalse/*假值*/;Xdot_Flag_Locking/*输入变化量标志锁存*/ = FlagTrue/*真值*/;CNT_Xdot/*计数器输入变化量*/ = 0;}
    settings: description=本路径的判据/动作：{X_Out = X_pre;X_Flag_Locking = FlagFalse;Xdot_Flag_Locking = FlagTrue;CNT_Xdot = 0;}。执行次序1；条件成立才执行本箭头动作。
  (junction 190) -> (junction 194) [order 1] : [(FlagTrue/*真值*/ == Xdot_Flag_Locking/*输入变化量标志锁存*/)&&((X/*自变量或输入量*/-Xin_pre/*输入量前一周期*/) < Xdot_CancelLim/*输入变化量解除限值*/)&&((X/*自变量或输入量*/-Xin_pre/*输入量前一周期*/) > -Xdot_CancelLim/*输入变化量解除限值*/)]
    settings: description=本路径的判据/动作：[(FlagTrue == Xdot_Flag_Locking)&&((X-Xin_pre) < Xdot_CancelLim)&&((X-Xin_pre) > -Xdot_CancelLim)]。执行次序1；条件成立才执行本箭头动作。
  (junction 190) -> (junction 15) [order 2] : {X_Out/*自变量或输入量输出*/ = X/*自变量或输入量*/;X_Flag_Locking/*自变量或输入量标志锁存*/ = FlagFalse/*假值*/;Xdot_Flag_Locking/*输入变化量标志锁存*/ = FlagFalse/*假值*/;CNT_Xdot/*计数器输入变化量*/ = 0;CNT_X/*计数器自变量或输入量*/ = 0;}
    settings: description=本路径的判据/动作：{X_Out = X;X_Flag_Locking = FlagFalse;Xdot_Flag_Locking = FlagFalse;CNT_Xdot = 0;CNT_X = 0;}。执行次序2；条件成立才执行本箭头动作。
  (junction 194) -> (junction 198) : {CNT_Xdot/*计数器输入变化量*/++;}
    settings: description=本路径的判据/动作：{CNT_Xdot++;}。执行次序1；条件成立才执行本箭头动作。
  (junction 216) -> (junction 230) [order 1] : [CNT_X/*计数器自变量或输入量*/ > 5]
    settings: description=本路径的判据/动作：[CNT_X > 5]。执行次序1；条件成立才执行本箭头动作。
  (junction 216) -> (junction 148) [order 2] : {X_Out/*自变量或输入量输出*/ = X_pre/*自变量或输入量前一周期*/;X_Flag_Locking/*自变量或输入量标志锁存*/ = FlagTrue/*真值*/;Xdot_Flag_Locking/*输入变化量标志锁存*/ = FlagFalse/*假值*/;}
    settings: description=本路径的判据/动作：{X_Out = X_pre;X_Flag_Locking = FlagTrue;Xdot_Flag_Locking = FlagFalse;}。执行次序2；条件成立才执行本箭头动作。
  (junction 230) -> (junction 218) : {X_Out/*自变量或输入量输出*/ = X/*自变量或输入量*/;X_Flag_Locking/*自变量或输入量标志锁存*/ = FlagFalse/*假值*/;Xdot_Flag_Locking/*输入变化量标志锁存*/ = FlagFalse/*假值*/;}
    settings: description=本路径的判据/动作：{X_Out = X;X_Flag_Locking = FlagFalse;Xdot_Flag_Locking = FlagFalse;}。执行次序1；条件成立才执行本箭头动作。
  (junction 198) -> (junction 197) [order 1] : [CNT_Xdot/*计数器输入变化量*/ > Xdot_Cancelcycle/*输入变化量解除确认周期数*/]
    settings: description=本路径的判据/动作：[CNT_Xdot > Xdot_Cancelcycle]。执行次序1；条件成立才执行本箭头动作。
  (junction 198) -> (junction 107) [order 2] : {X_Out/*自变量或输入量输出*/ = X_pre/*自变量或输入量前一周期*/;X_Flag_Locking/*自变量或输入量标志锁存*/ = FlagFalse/*假值*/;Xdot_Flag_Locking/*输入变化量标志锁存*/ = FlagTrue/*真值*/;}
    settings: description=本路径的判据/动作：{X_Out = X_pre;X_Flag_Locking = FlagFalse;Xdot_Flag_Locking = FlagTrue;}。执行次序2；条件成立才执行本箭头动作。
  (junction 197) -> (junction 196) : {X_Out/*自变量或输入量输出*/ = X/*自变量或输入量*/;X_Flag_Locking/*自变量或输入量标志锁存*/ = FlagFalse/*假值*/;Xdot_Flag_Locking/*输入变化量标志锁存*/ = FlagFalse/*假值*/;}
    settings: description=本路径的判据/动作：{X_Out = X;X_Flag_Locking = FlagFalse;Xdot_Flag_Locking = FlagFalse;}。执行次序1；条件成立才执行本箭头动作。
  (junction 107) -> (junction 15)
    settings: description=无附加条件的迁移路径，执行次序1；沿本图当前连接推进。
  (junction 196) -> (junction 107)
    settings: description=无附加条件的迁移路径，执行次序1；沿本图当前连接推进。
  (junction 187) -> (junction 196)
    settings: description=无附加条件的迁移路径，执行次序1；沿本图当前连接推进。
  (junction 148) -> (junction 187)
    settings: description=无附加条件的迁移路径，执行次序1；沿本图当前连接推进。
  (junction 240) -> (junction 218)
    settings: description=无附加条件的迁移路径，执行次序1；沿本图当前连接推进。
  (junction 218) -> (junction 148)
    settings: description=无附加条件的迁移路径，执行次序1；沿本图当前连接推进。
  (junction 15) -> (junction 83)
    settings: description=无附加条件的迁移路径，执行次序1；沿本图当前连接推进。
  data: X input single; Xin_pre input single; X_ulim input single; X_llim input single =0; X_Flag_Locking output boolean =0; Xdot_Flag_Locking output boolean =0; Xdot_lim input single; FlagTrue local boolean =1; Xdot_CancelLim input single; Xdot_Cancelcycle input single; X_Out output single =0; CNT_X local uint32 =0; X_pre input single; FlagFalse local boolean =0; CNT_Xdot local uint32 =0

== stateflow chart turbo_controller/CLM/Stop/Stop_Control ==
  note: 停车中的油路关闭、电机拖转和完成判断
      |
      | 接收停车命令、排温T4、转速Nc、原运行状态及Time_ms。StopZero分支直接置停车完成并关闭电机；
      | 普通停车先按约1 s等待条件处理阀门与供油。
      |
      | 图内对Nc≤7000、T4≥100设置了电机开通50的拖转路径，并限制拖转计时为约15 s；还存在低温、低
      | 转速和不同运行状态的提前完成路径。条件按图上的分支顺序判断，不能把所有温度与转速比较拼成一
      | 个同时成立的条件。
      |
      | 计时门限为等待毫秒数/Time_ms，例如Time_ms=20时15 s对应750次调用。输出是电机、油阀及Stop_Fi
      | nish，随后分别进入板级输出和发动机状态转换。
  (default) -> (junction 950)
    settings: description=无附加条件的迁移路径，执行次序1；沿本图当前连接推进。
  (junction 950) -> (junction 998) [order 1] : [StopZero/*停车零*/==true/*真值*/]
    settings: description=本路径的判据/动作：[StopZero==true]。执行次序1；条件成立才执行本箭头动作。
  (junction 950) -> (junction 956) [order 2]
    settings: description=无附加条件的迁移路径，执行次序2；沿本图当前连接推进。
  (junction 998) -> (junction 1000) : {StopFinish/*停车完成*/ = true/*真值*/;
      | Motor_Open/*起动电机开通计数*/ = 0;}
    settings: description=本路径的判据/动作：{StopFinish = true; Motor_Open = 0;}。执行次序1；条件成立才执行本箭头动作。
  (junction 958) -> (junction 962) [order 1] : [CNT_Wait/*计数器等待*/  >= (1000/Time_ms/*时间毫秒*/)]
    settings: description=本路径的判据/动作：[CNT_Wait >= (1000/Time_ms)]。执行次序1；条件成立才执行本箭头动作。
  (junction 956) -> (junction 958) [order 1] : [Flag_RunState/*标志运行状态*/~=4]
    settings: description=本路径的判据/动作：[Flag_RunState~=4]。执行次序1；条件成立才执行本箭头动作。
  (junction 962) -> (junction 960) : {EValve_Enable/*主油阀驱动使能*/=0;
      | Eblast_Enable/*副油阀驱动使能*/=0;
      | EValve_Open/*主油阀开通计数（每计数2毫秒）*/=0;
      | Eblast_Open/*副油阀开通计数（每计数2毫秒）*/=0;}
    settings: description=本路径的判据/动作：{EValve_Enable=0; Eblast_Enable=0; EValve_Open=0; Eblast_Open=0;}。执行次序1；条件成立才执行本箭头动作。
  (junction 958) -> (junction 960) [order 2] : {Accelerator/*油门／油泵给定控制量*/=0;
      | EValve_Enable/*主油阀驱动使能*/=1;
      | EValve_Open/*主油阀开通计数（每计数2毫秒）*/=30;
      | Eblast_Enable/*副油阀驱动使能*/=1;
      | Eblast_Open/*副油阀开通计数（每计数2毫秒）*/=30;}
    settings: description=本路径的判据/动作：{Accelerator=0; EValve_Enable=1; EValve_Open=30; Eblast_Enable=1; Eblast_Open=30;}。执行次序2；条件成立才执行本箭头动作。
  (junction 956) -> (junction 910) [order 2] : {StopFinish/*停车完成*/ = true/*真值*/;
      | Motor_Open/*起动电机开通计数*/ = uint16/*十六位无符号整数*/(0);}
    settings: description=本路径的判据/动作：{StopFinish = true; Motor_Open = uint16(0);}。执行次序2；条件成立才执行本箭头动作。
  (junction 960) -> (junction 979) [order 1] : [Nc/*发动机反馈转速（转每分）*/<=7000 & T4/*排气温度（℃）*/>=100]
    settings: description=本路径的判据/动作：[Nc<=7000 & T4>=100]。执行次序1；条件成立才执行本箭头动作。
  (junction 979) -> (junction 973) [order 1] : [CNT_Motor/*计数器电机*/ >= (15000/Time_ms/*时间毫秒*/)]
    settings: description=本路径的判据/动作：[CNT_Motor >= (15000/Time_ms)]。执行次序1；条件成立才执行本箭头动作。
  (junction 973) -> (junction 987) : {StopFinish/*停车完成*/ = true/*真值*/;
      | Motor_Open/*起动电机开通计数*/ = 0;}
    settings: description=本路径的判据/动作：{StopFinish = true; Motor_Open = 0;}。执行次序1；条件成立才执行本箭头动作。
  (junction 960) -> (junction 990) [order 2]
    settings: description=无附加条件的迁移路径，执行次序2；沿本图当前连接推进。
  (junction 979) -> (junction 983) [order 2] : {Motor_Open/*起动电机开通计数*/ = 50;
      | CNT_Motor/*计数器电机*/++;}
    settings: description=本路径的判据/动作：{Motor_Open = 50; CNT_Motor++;}。执行次序2；条件成立才执行本箭头动作。
  (junction 990) -> (junction 992) [order 1] : [T4/*排气温度（℃）*/<=100 ||  Nc/*发动机反馈转速（转每分）*/<=7000]
    settings: description=本路径的判据/动作：[T4<=100 || Nc<=7000]。执行次序1；条件成立才执行本箭头动作。
  (junction 990) -> (junction 978) [order 2]
    settings: description=无附加条件的迁移路径，执行次序2；沿本图当前连接推进。
  (junction 992) -> (junction 994) : {StopFinish/*停车完成*/ = true/*真值*/;
      | Motor_Open/*起动电机开通计数*/ = 0;}
    settings: description=本路径的判据/动作：{StopFinish = true; Motor_Open = 0;}。执行次序1；条件成立才执行本箭头动作。
  (junction 978) -> (junction 910) : {CNT_Wait/*计数器等待*/++;}
    settings: description=本路径的判据/动作：{CNT_Wait++;}。执行次序1；条件成立才执行本箭头动作。
  (junction 994) -> (junction 978)
    settings: description=无附加条件的迁移路径，执行次序1；沿本图当前连接推进。
  (junction 983) -> (junction 994)
    settings: description=无附加条件的迁移路径，执行次序1；沿本图当前连接推进。
  (junction 987) -> (junction 983)
    settings: description=无附加条件的迁移路径，执行次序1；沿本图当前连接推进。
  (junction 1000) -> (junction 987)
    settings: description=无附加条件的迁移路径，执行次序1；沿本图当前连接推进。
  (junction 910) -> (junction 952)
    settings: description=无附加条件的迁移路径，执行次序1；沿本图当前连接推进。
  data: Time_ms input single; Nc input single; T4 input single; StopZero input boolean; Accelerator output single =0; EValve_Open output uint16 =0; Eblast_Open output uint16 =0; Motor_Open output uint16 =0; EValve_Enable output uint8 =0; Eblast_Enable output uint8 =0; StopFinish output uint8 =0; CNT_Wait local uint32 =0; Flag_RunState input uint8; CNT_Motor local uint32 =0

== stateflow chart turbo_controller/COMMRead_ISM/ISM/Subsystem2/Xlim_Xdot_Judge ==
  note: 排温超限标志怎样置位和解除
      |
      | 父级给本图三个量：本次排温X、上限X_ulim=930 ℃、上次接受的温度X_pre。本图有记忆，既判断当
      | 前值，也记住故障状态和恢复次数。
      |
      | 当X超过上限时，置X_Flag_Locking=true，温度输出X_Out采用X_pre，并清恢复计数。这样一次异常不
      | 会覆盖内部保留的有效温度。
      | 当X重新回到允许上限内时，开始累计CNT_X；连续确认到CNT_X>5后，接受当前X并解除故障标志。确认
      | 未完成时沿图中的保持路径继续处理。
      |
      | 这里的“5”是调用次数，不是5秒；本工程控制周期Ts_ms为20 ms。确切解除时刻还受先计数还是先比
      | 较的路径顺序影响。
      |
      | 输出故障标志交给Sensor总线，温度输出仅供本图下一次保持。未使用的Xin_pre和突变计数已删除，
      | 因此不要把它解释成温度变化率故障检测。
  (default) -> (junction 232)
    settings: description=无附加条件的迁移路径，执行次序1；沿本图当前连接推进。
  (junction 232) -> (junction 234) [order 1] : [X/*自变量或输入量*/ > X_ulim/*输入上限*/]
    settings: description=本路径的判据/动作：[X > X_ulim]。执行次序1；条件成立才执行本箭头动作。
  (junction 232) -> (junction 33) [order 2]
    settings: description=无附加条件的迁移路径，执行次序2；沿本图当前连接推进。
  (junction 234) -> (junction 240) : {X_Out/*自变量或输入量输出*/ = X_pre/*自变量或输入量前一周期*/;X_Flag_Locking/*自变量或输入量标志锁存*/ = FlagTrue/*真值*/;CNT_X/*计数器自变量或输入量*/ = 0;}
    settings: description=本路径的判据/动作：{X_Out = X_pre;X_Flag_Locking = FlagTrue;CNT_X = 0;}。执行次序1；条件成立才执行本箭头动作。
  (junction 33) -> (junction 146) [order 1] : [(X_Flag_Locking/*自变量或输入量标志锁存*/ == FlagTrue/*真值*/) && (X/*自变量或输入量*/<= X_ulim/*输入上限*/) ]
    settings: description=本路径的判据/动作：[(X_Flag_Locking == FlagTrue) && (X<= X_ulim) ]。执行次序1；条件成立才执行本箭头动作。
  (junction 33) -> (junction 15) [order 2] : {X_Out/*自变量或输入量输出*/ = X/*自变量或输入量*/;X_Flag_Locking/*自变量或输入量标志锁存*/ = FlagFalse/*假值*/;CNT_X/*计数器自变量或输入量*/ = 0;}
    settings: description=本路径的判据/动作：{X_Out = X;X_Flag_Locking = FlagFalse;CNT_X = 0;}。执行次序2；条件成立才执行本箭头动作。
  (junction 146) -> (junction 216) : {CNT_X/*计数器自变量或输入量*/++;}
    settings: description=本路径的判据/动作：{CNT_X++;}。执行次序1；条件成立才执行本箭头动作。
  (junction 216) -> (junction 230) [order 1] : [CNT_X/*计数器自变量或输入量*/ > 5]
    settings: description=本路径的判据/动作：[CNT_X > 5]。执行次序1；条件成立才执行本箭头动作。
  (junction 216) -> (junction 148) [order 2] : {X_Out/*自变量或输入量输出*/ = X_pre/*自变量或输入量前一周期*/;X_Flag_Locking/*自变量或输入量标志锁存*/ = FlagTrue/*真值*/;}
    settings: description=本路径的判据/动作：{X_Out = X_pre;X_Flag_Locking = FlagTrue;}。执行次序2；条件成立才执行本箭头动作。
  (junction 230) -> (junction 218) : {X_Out/*自变量或输入量输出*/ = X/*自变量或输入量*/;X_Flag_Locking/*自变量或输入量标志锁存*/ = FlagFalse/*假值*/;}
    settings: description=本路径的判据/动作：{X_Out = X;X_Flag_Locking = FlagFalse;}。执行次序1；条件成立才执行本箭头动作。
  (junction 240) -> (junction 218)
    settings: description=无附加条件的迁移路径，执行次序1；沿本图当前连接推进。
  (junction 148) -> (junction 15)
    settings: description=无附加条件的迁移路径，执行次序1；沿本图当前连接推进。
  (junction 218) -> (junction 148)
    settings: description=无附加条件的迁移路径，执行次序1；沿本图当前连接推进。
  (junction 15) -> (junction 83)
    settings: description=无附加条件的迁移路径，执行次序1；沿本图当前连接推进。
  data: X input single; X_ulim input single; X_Flag_Locking output boolean =0; FlagTrue local boolean =1; X_Out output single =0; CNT_X local uint32 =0; X_pre input single; FlagFalse local boolean =0

== stateflow chart turbo_controller/CLM/Start/Range ==
  note: 本实例把普通起动图产生的Accelerator限制在0～5000，输出为起动泵控制编码。图内算出的曲线即使
      | 大于5000也会在此截住。
      |
      | 把一个数限制在允许范围内
      |
      | 输入包括待处理值、允许下限和允许上限。先比较是否越过上限，越过就输出上限；未超过上限时再检
      | 查下限，小于下限就输出下限；落在范围内则原样通过。恰好等于边界的值也保留。
      |
      | 计算式：输出 = min(max(输入，下限)，上限)。
      | 例如下限为0、上限为100时，输入120输出100，输入-5输出0，输入60输出60。这里不做平均、不计算
      | 变化速度，也不记住上一拍；它只防止当前数值越界。具体边界由父子系统连入，不能把此处的输出一
      | 律理解为百分比。
  (default) -> (junction 6)
    settings: description=无附加条件的迁移路径，执行次序1；沿本图当前连接推进。
  (junction 6) -> (junction 7) [order 1] : [In/*输入*/ <= Min/*下限*/]
    settings: description=本路径的判据/动作：[In <= Min]。执行次序1；条件成立才执行本箭头动作。
  (junction 6) -> (junction 29) [order 2] : {Out/*输出*/ = In/*输入*/;}
    settings: description=本路径的判据/动作：{Out = In;}。执行次序2；条件成立才执行本箭头动作。
  (junction 7) -> (junction 11) : {Out/*输出*/ = Min/*下限*/;}
    settings: description=本路径的判据/动作：{Out = Min;}。执行次序1；条件成立才执行本箭头动作。
  (junction 11) -> (junction 29)
    settings: description=无附加条件的迁移路径，执行次序1；沿本图当前连接推进。
  (junction 29) -> (junction 13)
    settings: description=无附加条件的迁移路径，执行次序1；沿本图当前连接推进。
  (junction 13) -> (junction 15) [order 1] : [Out/*输出*/ >= Max/*上限*/]
    settings: description=本路径的判据/动作：[Out >= Max]。执行次序1；条件成立才执行本箭头动作。
  (junction 13) -> (junction 20) [order 2]
    settings: description=无附加条件的迁移路径，执行次序2；沿本图当前连接推进。
  (junction 15) -> (junction 17) : {Out/*输出*/ = Max/*上限*/;}
    settings: description=本路径的判据/动作：{Out = Max;}。执行次序1；条件成立才执行本箭头动作。
  (junction 17) -> (junction 20)
    settings: description=无附加条件的迁移路径，执行次序1；沿本图当前连接推进。
  (junction 20) -> (junction 25)
    settings: description=无附加条件的迁移路径，执行次序1；沿本图当前连接推进。
  data: In input single; Max input single; Min input single; Out output single =0

== stateflow chart turbo_controller/CLM/Start/Subsystem/Timmer_ms ==
  note: 起动参数切换所用的毫秒定时器
      |
      | 每次调用按Ts_ms所代表的时间推进计数，到Time_ms对应的调用次数时输出到时状态。当前控制节拍20
      |  ms，1000 ms要累计50次调用，不能把内部计数50理解为50 s。
      |
      | 父系统利用此状态决定继续沿用历史参数，还是切换到本次压力计算的参数。这里不读取压力，也不决
      | 定m1、m2等曲线值；它只提供参数切换的时间条件。
  (default) -> (junction 26)
    settings: description=无附加条件的迁移路径，执行次序1；沿本图当前连接推进。
  (junction 26) -> (junction 3) [order 1] : [true/*真值*/ == In/*输入*/]
    settings: description=本路径的判据/动作：[true == In]。执行次序1；条件成立才执行本箭头动作。
  (junction 3) -> (junction 5) [order 1] : [Cnt/*计数器*/ >= uint32/*三十二位无符号整数*/(100000)]
    settings: description=本路径的判据/动作：[Cnt >= uint32(100000)]。执行次序1；条件成立才执行本箭头动作。
  (junction 26) -> (junction 43) [order 2] : {Cnt/*计数器*/ = 0;Out/*输出*/ = 0;}
    settings: description=本路径的判据/动作：{Cnt = 0;Out = 0;}。执行次序2；条件成立才执行本箭头动作。
  (junction 3) -> (junction 10) [order 2] : {Cnt/*计数器*/++;}
    settings: description=本路径的判据/动作：{Cnt++;}。执行次序2；条件成立才执行本箭头动作。
  (junction 5) -> (junction 12) : {Cnt/*计数器*/ = 100000;}
    settings: description=本路径的判据/动作：{Cnt = 100000;}。执行次序1；条件成立才执行本箭头动作。
  (junction 12) -> (junction 10)
    settings: description=无附加条件的迁移路径，执行次序1；沿本图当前连接推进。
  (junction 10) -> (junction 30)
    settings: description=无附加条件的迁移路径，执行次序1；沿本图当前连接推进。
  (junction 30) -> (junction 33) [order 1] : [Cnt/*计数器*/ >uint32/*三十二位无符号整数*/(Time_ms/*时间毫秒*//Ts_ms/*采样周期毫秒*/)]
    settings: description=本路径的判据/动作：[Cnt >uint32(Time_ms/Ts_ms)]。执行次序1；条件成立才执行本箭头动作。
  (junction 30) -> (junction 37) [order 2] : {Out/*输出*/ = 0;}
    settings: description=本路径的判据/动作：{Out = 0;}。执行次序2；条件成立才执行本箭头动作。
  (junction 33) -> (junction 36) : {Out/*输出*/ = 1;}
    settings: description=本路径的判据/动作：{Out = 1;}。执行次序1；条件成立才执行本箭头动作。
  (junction 36) -> (junction 37)
    settings: description=无附加条件的迁移路径，执行次序1；沿本图当前连接推进。
  (junction 37) -> (junction 55)
    settings: description=无附加条件的迁移路径，执行次序1；沿本图当前连接推进。
  (junction 55) -> (junction 43)
    settings: description=无附加条件的迁移路径，执行次序1；沿本图当前连接推进。
  (junction 43) -> (junction 71)
    settings: description=无附加条件的迁移路径，执行次序1；沿本图当前连接推进。
  data: Cnt local uint32 =0; Out output uint8 =0; In input boolean; Time_ms input single; Ts_ms parameter single

== stateflow chart turbo_controller/CLM/Start/Subsystem/Hold ==
  note: 识别本次执行的第一次调用
      |
      | 内部保持一个首次标志。第一次进入时给出用于初始化的标志，之后把内部状态切换为已经执行，使后
      | 续调用采用保持或正常处理路径。
      |
      | 本图自身不存储温度、油压或参数数组。需要保留的具体数值在父系统的开关与延迟中保存；本图只告
      | 诉父系统何时取初值。它也不是每拍都产生一次上升沿。重新初始化模型时会重新开始这一首次判断。
  (default) -> (junction 26)
    settings: description=无附加条件的迁移路径，执行次序1；沿本图当前连接推进。
  (junction 26) -> (junction 3) [order 1] : [true/*真值*/ == Flag_First/*标志首次*/]
    settings: description=本路径的判据/动作：[true == Flag_First]。执行次序1；条件成立才执行本箭头动作。
  (junction 26) -> (junction 43) [order 2] : {Out/*输出*/ = true/*真值*/;
      | Flag_First/*标志首次*/ = true/*真值*/;}
    settings: description=本路径的判据/动作：{Out = true; Flag_First = true;}。执行次序2；条件成立才执行本箭头动作。
  (junction 3) -> (junction 55) : {Out/*输出*/ = false/*假值*/;}
    settings: description=本路径的判据/动作：{Out = false;}。执行次序1；条件成立才执行本箭头动作。
  (junction 55) -> (junction 43)
    settings: description=无附加条件的迁移路径，执行次序1；沿本图当前连接推进。
  (junction 43) -> (junction 71)
    settings: description=无附加条件的迁移路径，执行次序1；沿本图当前连接推进。
  data: Out output boolean =0; Flag_First local boolean =0

== stateflow chart turbo_controller/CLM/ClpControl/CtrlLaw/Range1 ==
  note: 本实例把通信入口总压P1t_calc限制在30～100，再除以100得到PI步长修正系数q。例如入口总压20先
      | 变30，q=0.3；入口总压80得到q=0.8。
      |
      | 把一个数限制在允许范围内
      |
      | 输入包括待处理值、允许下限和允许上限。先比较是否越过上限，越过就输出上限；未超过上限时再检
      | 查下限，小于下限就输出下限；落在范围内则原样通过。恰好等于边界的值也保留。
      |
      | 计算式：输出 = min(max(输入，下限)，上限)。
      | 例如下限为0、上限为100时，输入120输出100，输入-5输出0，输入60输出60。这里不做平均、不计算
      | 变化速度，也不记住上一拍；它只防止当前数值越界。具体边界由父子系统连入，不能把此处的输出一
      | 律理解为百分比。
  (default) -> (junction 6)
    settings: description=无附加条件的迁移路径，执行次序1；沿本图当前连接推进。
  (junction 6) -> (junction 7) [order 1] : [In/*输入*/ <= Min/*下限*/]
    settings: description=本路径的判据/动作：[In <= Min]。执行次序1；条件成立才执行本箭头动作。
  (junction 6) -> (junction 29) [order 2] : {Out/*输出*/ = In/*输入*/;}
    settings: description=本路径的判据/动作：{Out = In;}。执行次序2；条件成立才执行本箭头动作。
  (junction 7) -> (junction 11) : {Out/*输出*/ = Min/*下限*/;}
    settings: description=本路径的判据/动作：{Out = Min;}。执行次序1；条件成立才执行本箭头动作。
  (junction 11) -> (junction 29)
    settings: description=无附加条件的迁移路径，执行次序1；沿本图当前连接推进。
  (junction 29) -> (junction 13)
    settings: description=无附加条件的迁移路径，执行次序1；沿本图当前连接推进。
  (junction 13) -> (junction 15) [order 1] : [Out/*输出*/ >= Max/*上限*/]
    settings: description=本路径的判据/动作：[Out >= Max]。执行次序1；条件成立才执行本箭头动作。
  (junction 13) -> (junction 20) [order 2]
    settings: description=无附加条件的迁移路径，执行次序2；沿本图当前连接推进。
  (junction 15) -> (junction 17) : {Out/*输出*/ = Max/*上限*/;}
    settings: description=本路径的判据/动作：{Out = Max;}。执行次序1；条件成立才执行本箭头动作。
  (junction 17) -> (junction 20)
    settings: description=无附加条件的迁移路径，执行次序1；沿本图当前连接推进。
  (junction 20) -> (junction 25)
    settings: description=无附加条件的迁移路径，执行次序1；沿本图当前连接推进。
  data: In input single; Max input single; Min input single; Out output single =0

== stateflow chart turbo_controller/CLM/ClpControl/CtrlLaw/Range ==
  note: 本实例限制PI每拍计算的泵给定增量，上下限为±10×q，其中q=限幅后的入口总压/100，q在0.3～1之间
      | 。例如q=0.5时只允许本拍增加或减少5。
      |
      | 把一个数限制在允许范围内
      |
      | 输入包括待处理值、允许下限和允许上限。先比较是否越过上限，越过就输出上限；未超过上限时再检
      | 查下限，小于下限就输出下限；落在范围内则原样通过。恰好等于边界的值也保留。
      |
      | 计算式：输出 = min(max(输入，下限)，上限)。
      | 例如下限为0、上限为100时，输入120输出100，输入-5输出0，输入60输出60。这里不做平均、不计算
      | 变化速度，也不记住上一拍；它只防止当前数值越界。具体边界由父子系统连入，不能把此处的输出一
      | 律理解为百分比。
  (default) -> (junction 6)
    settings: description=无附加条件的迁移路径，执行次序1；沿本图当前连接推进。
  (junction 6) -> (junction 7) [order 1] : [In/*输入*/ <= Min/*下限*/]
    settings: description=本路径的判据/动作：[In <= Min]。执行次序1；条件成立才执行本箭头动作。
  (junction 6) -> (junction 29) [order 2] : {Out/*输出*/ = In/*输入*/;}
    settings: description=本路径的判据/动作：{Out = In;}。执行次序2；条件成立才执行本箭头动作。
  (junction 7) -> (junction 11) : {Out/*输出*/ = Min/*下限*/;}
    settings: description=本路径的判据/动作：{Out = Min;}。执行次序1；条件成立才执行本箭头动作。
  (junction 11) -> (junction 29)
    settings: description=无附加条件的迁移路径，执行次序1；沿本图当前连接推进。
  (junction 29) -> (junction 13)
    settings: description=无附加条件的迁移路径，执行次序1；沿本图当前连接推进。
  (junction 13) -> (junction 15) [order 1] : [Out/*输出*/ >= Max/*上限*/]
    settings: description=本路径的判据/动作：[Out >= Max]。执行次序1；条件成立才执行本箭头动作。
  (junction 13) -> (junction 20) [order 2]
    settings: description=无附加条件的迁移路径，执行次序2；沿本图当前连接推进。
  (junction 15) -> (junction 17) : {Out/*输出*/ = Max/*上限*/;}
    settings: description=本路径的判据/动作：{Out = Max;}。执行次序1；条件成立才执行本箭头动作。
  (junction 17) -> (junction 20)
    settings: description=无附加条件的迁移路径，执行次序1；沿本图当前连接推进。
  (junction 20) -> (junction 25)
    settings: description=无附加条件的迁移路径，执行次序1；沿本图当前连接推进。
  data: In input single; Max input single; Min input single; Out output single =0

== stateflow chart turbo_controller/COMMRead_ISM/ISM/Calibrating_T0/Range ==
  note: 本实例限制T0在-70～175 ℃。总温编码减80后若为9999等大值，最终显示175；这属于上限截断，不代
      | 表真实温度就是175 ℃，本处未另行产生总温故障标志。
      |
      | 把一个数限制在允许范围内
      |
      | 输入包括待处理值、允许下限和允许上限。先比较是否越过上限，越过就输出上限；未超过上限时再检
      | 查下限，小于下限就输出下限；落在范围内则原样通过。恰好等于边界的值也保留。
      |
      | 计算式：输出 = min(max(输入，下限)，上限)。
      | 例如下限为0、上限为100时，输入120输出100，输入-5输出0，输入60输出60。这里不做平均、不计算
      | 变化速度，也不记住上一拍；它只防止当前数值越界。具体边界由父子系统连入，不能把此处的输出一
      | 律理解为百分比。
  (default) -> (junction 6)
    settings: description=无附加条件的迁移路径，执行次序1；沿本图当前连接推进。
  (junction 6) -> (junction 7) [order 1] : [In/*输入*/ <= Min/*下限*/]
    settings: description=本路径的判据/动作：[In <= Min]。执行次序1；条件成立才执行本箭头动作。
  (junction 6) -> (junction 29) [order 2] : {Out/*输出*/ = In/*输入*/;}
    settings: description=本路径的判据/动作：{Out = In;}。执行次序2；条件成立才执行本箭头动作。
  (junction 7) -> (junction 11) : {Out/*输出*/ = Min/*下限*/;}
    settings: description=本路径的判据/动作：{Out = Min;}。执行次序1；条件成立才执行本箭头动作。
  (junction 11) -> (junction 29)
    settings: description=无附加条件的迁移路径，执行次序1；沿本图当前连接推进。
  (junction 29) -> (junction 13)
    settings: description=无附加条件的迁移路径，执行次序1；沿本图当前连接推进。
  (junction 13) -> (junction 15) [order 1] : [Out/*输出*/ >= Max/*上限*/]
    settings: description=本路径的判据/动作：[Out >= Max]。执行次序1；条件成立才执行本箭头动作。
  (junction 13) -> (junction 20) [order 2]
    settings: description=无附加条件的迁移路径，执行次序2；沿本图当前连接推进。
  (junction 15) -> (junction 17) : {Out/*输出*/ = Max/*上限*/;}
    settings: description=本路径的判据/动作：{Out = Max;}。执行次序1；条件成立才执行本箭头动作。
  (junction 17) -> (junction 20)
    settings: description=无附加条件的迁移路径，执行次序1；沿本图当前连接推进。
  (junction 20) -> (junction 25)
    settings: description=无附加条件的迁移路径，执行次序1；沿本图当前连接推进。
  data: In input single; Max input single; Min input single; Out output single =0

== stateflow chart turbo_controller/COMMRead_ISM/ISM/HuanSuanN/Range ==
  note: 本实例把温度修正转速限制在0～75000 rpm。输出用于记录与回传；不是闭环PI所用的Nc_Filter。
      |
      | 把一个数限制在允许范围内
      |
      | 输入包括待处理值、允许下限和允许上限。先比较是否越过上限，越过就输出上限；未超过上限时再检
      | 查下限，小于下限就输出下限；落在范围内则原样通过。恰好等于边界的值也保留。
      |
      | 计算式：输出 = min(max(输入，下限)，上限)。
      | 例如下限为0、上限为100时，输入120输出100，输入-5输出0，输入60输出60。这里不做平均、不计算
      | 变化速度，也不记住上一拍；它只防止当前数值越界。具体边界由父子系统连入，不能把此处的输出一
      | 律理解为百分比。
  (default) -> (junction 6)
    settings: description=无附加条件的迁移路径，执行次序1；沿本图当前连接推进。
  (junction 6) -> (junction 7) [order 1] : [In/*输入*/ <= Min/*下限*/]
    settings: description=本路径的判据/动作：[In <= Min]。执行次序1；条件成立才执行本箭头动作。
  (junction 6) -> (junction 29) [order 2] : {Out/*输出*/ = In/*输入*/;}
    settings: description=本路径的判据/动作：{Out = In;}。执行次序2；条件成立才执行本箭头动作。
  (junction 7) -> (junction 11) : {Out/*输出*/ = Min/*下限*/;}
    settings: description=本路径的判据/动作：{Out = Min;}。执行次序1；条件成立才执行本箭头动作。
  (junction 11) -> (junction 29)
    settings: description=无附加条件的迁移路径，执行次序1；沿本图当前连接推进。
  (junction 29) -> (junction 13)
    settings: description=无附加条件的迁移路径，执行次序1；沿本图当前连接推进。
  (junction 13) -> (junction 15) [order 1] : [Out/*输出*/ >= Max/*上限*/]
    settings: description=本路径的判据/动作：[Out >= Max]。执行次序1；条件成立才执行本箭头动作。
  (junction 13) -> (junction 20) [order 2]
    settings: description=无附加条件的迁移路径，执行次序2；沿本图当前连接推进。
  (junction 15) -> (junction 17) : {Out/*输出*/ = Max/*上限*/;}
    settings: description=本路径的判据/动作：{Out = Max;}。执行次序1；条件成立才执行本箭头动作。
  (junction 17) -> (junction 20)
    settings: description=无附加条件的迁移路径，执行次序1；沿本图当前连接推进。
  (junction 20) -> (junction 25)
    settings: description=无附加条件的迁移路径，执行次序1；沿本图当前连接推进。
  data: In input single; Max input single; Min input single; Out output single =0

== stateflow chart turbo_controller/CLM/ControlOut_Manage/Accelerator_Manage/ServoCtrlOut ==
  note: 按当前控制模式选择并限制油泵给定
      |
      | EngineCtrlMode决定本次采用哪一种候选，不是比较几种候选谁最大。起动选Vin_Start，停车选Vin_S
      | top；不属于这些指定分支时走原位候选。
      |
      | 闭环模式选Vin_Idle，但先限制在CloseLoopMin～CloseLoopMax；手动模式选Vin_Manual，限制在Manu
      | alAccMin～ManualAccMax。
      | 通用限幅关系为输出=min(max(候选,下限),上限)。
      |
      | 每次选择还给出ServoCtrlFlag：例如闭环候选大于上限，就输出上限并标“闭环上限”；在范围内则
      | 标正常闭环。这样记录的不只是一个给定值，也能看出是否被限幅。
      |
      | 本图没有低通滤波，也不直接发送串口命令。输出回到Accelerator_Manage后，外层还可能按复位恢复
      | 工作标志选择恢复给定。
  (default) -> (junction 2)
    settings: description=无附加条件的迁移路径，执行次序1；沿本图当前连接推进。
  (junction 2) -> (junction 5) [order 2]
    settings: description=无附加条件的迁移路径，执行次序2；沿本图当前连接推进。
  (junction 5) -> (junction 9) [order 2]
    settings: description=无附加条件的迁移路径，执行次序2；沿本图当前连接推进。
  (junction 9) -> (junction 109) [order 1] : [PG_CtrlMode_CloseLoop/*闭合回路*/ == EngineCtrlMode/*发动机控制模式*/]
    settings: description=本路径的判据/动作：[PG_CtrlMode_CloseLoop == EngineCtrlMode]。执行次序1；条件成立才执行本箭头动作。
  (junction 109) -> (junction 114) [order 1] : [Vin_Idle/*输入电压或输入控制量慢车*/ >= CloseLoopMax/*闭合回路上限*/]
    settings: description=本路径的判据/动作：[Vin_Idle >= CloseLoopMax]。执行次序1；条件成立才执行本箭头动作。
  (junction 2) -> (junction 3) [order 1] : [PG_CtrlMode_Start/*起动*/ == EngineCtrlMode/*发动机控制模式*/]
    settings: description=本路径的判据/动作：[PG_CtrlMode_Start == EngineCtrlMode]。执行次序1；条件成立才执行本箭头动作。
  (junction 5) -> (junction 7) [order 1] : [PG_CtrlMode_ManualAcc/*手动油门*/ == EngineCtrlMode/*发动机控制模式*/]
    settings: description=本路径的判据/动作：[PG_CtrlMode_ManualAcc == EngineCtrlMode]。执行次序1；条件成立才执行本箭头动作。
  (junction 9) -> (junction 146) [order 2]
    settings: description=无附加条件的迁移路径，执行次序2；沿本图当前连接推进。
  (junction 109) -> (junction 126) [order 2]
    settings: description=无附加条件的迁移路径，执行次序2；沿本图当前连接推进。
  (junction 114) -> (junction 130) : {Vout/*输出电压或输出控制量*/ =CloseLoopMax/*闭合回路上限*/;
      |  ServoCtrlFlag/*油泵给定选择标志*/ = PG_ServoCtrlMode_CloseLoopMax/*闭合回路上限*/;}
    settings: description=本路径的判据/动作：{Vout =CloseLoopMax; ServoCtrlFlag = PG_ServoCtrlMode_CloseLoopMax;}。执行次序1；条件成立才执行本箭头动作。
  (junction 146) -> (junction 26) [order 2] : {Vout/*输出电压或输出控制量*/ = Vin_Origin/*输入电压或输入控制量原位*/;
      |  ServoCtrlFlag/*油泵给定选择标志*/ = PG_CtrlMode_Origin/*原位*/;}
    settings: description=本路径的判据/动作：{Vout = Vin_Origin; ServoCtrlFlag = PG_CtrlMode_Origin;}。执行次序2；条件成立才执行本箭头动作。
  (junction 26) -> (junction 30)
    settings: description=无附加条件的迁移路径，执行次序1；沿本图当前连接推进。
  (junction 126) -> (junction 131) [order 1] : [Vin_Idle/*输入电压或输入控制量慢车*/ <= CloseLoopMin/*闭合回路下限*/]
    settings: description=本路径的判据/动作：[Vin_Idle <= CloseLoopMin]。执行次序1；条件成立才执行本箭头动作。
  (junction 146) -> (junction 148) [order 1] : [PG_CtrlMode_Stop/*停车*/ == EngineCtrlMode/*发动机控制模式*/]
    settings: description=本路径的判据/动作：[PG_CtrlMode_Stop == EngineCtrlMode]。执行次序1；条件成立才执行本箭头动作。
  (junction 150) -> (junction 26)
    settings: description=无附加条件的迁移路径，执行次序1；沿本图当前连接推进。
  (junction 126) -> (junction 127) [order 2] : {Vout/*输出电压或输出控制量*/ =Vin_Idle/*输入电压或输入控制量慢车*/;
      |  ServoCtrlFlag/*油泵给定选择标志*/ = PG_ServoCtrlMode_CloseLoop/*闭合回路*/;}
    settings: description=本路径的判据/动作：{Vout =Vin_Idle; ServoCtrlFlag = PG_ServoCtrlMode_CloseLoop;}。执行次序2；条件成立才执行本箭头动作。
  (junction 131) -> (junction 123) : {Vout/*输出电压或输出控制量*/ =CloseLoopMin/*闭合回路下限*/;
      |  ServoCtrlFlag/*油泵给定选择标志*/ = PG_ServoCtrlMode_CloseLoopMin/*闭合回路下限*/;}
    settings: description=本路径的判据/动作：{Vout =CloseLoopMin; ServoCtrlFlag = PG_ServoCtrlMode_CloseLoopMin;}。执行次序1；条件成立才执行本箭头动作。
  (junction 148) -> (junction 150) : {Vout/*输出电压或输出控制量*/ = Vin_Stop/*输入电压或输入控制量停车*/;
      |  ServoCtrlFlag/*油泵给定选择标志*/ = PG_CtrlMode_Stop/*停车*/;}
    settings: description=本路径的判据/动作：{Vout = Vin_Stop; ServoCtrlFlag = PG_CtrlMode_Stop;}。执行次序1；条件成立才执行本箭头动作。
  (junction 127) -> (junction 150)
    settings: description=无附加条件的迁移路径，执行次序1；沿本图当前连接推进。
  (junction 123) -> (junction 127)
    settings: description=无附加条件的迁移路径，执行次序1；沿本图当前连接推进。
  (junction 130) -> (junction 123)
    settings: description=无附加条件的迁移路径，执行次序1；沿本图当前连接推进。
  (junction 105) -> (junction 130)
    settings: description=无附加条件的迁移路径，执行次序1；沿本图当前连接推进。
  (junction 7) -> (junction 92) [order 2]
    settings: description=无附加条件的迁移路径，执行次序2；沿本图当前连接推进。
  (junction 92) -> (junction 105) [order 2] : {Vout/*输出电压或输出控制量*/ =Vin_Manual/*输入电压或输入控制量手动*/;
      |  ServoCtrlFlag/*油泵给定选择标志*/ = PG_ServoCtrlMode_ManualAcc/*手动油门*/;}
    settings: description=本路径的判据/动作：{Vout =Vin_Manual; ServoCtrlFlag = PG_ServoCtrlMode_ManualAcc;}。执行次序2；条件成立才执行本箭头动作。
  (junction 7) -> (junction 93) [order 1] : [Vin_Manual/*输入电压或输入控制量手动*/ >= ManualAccMax/*手动油门上限*/]
    settings: description=本路径的判据/动作：[Vin_Manual >= ManualAccMax]。执行次序1；条件成立才执行本箭头动作。
  (junction 92) -> (junction 96) [order 1] : [Vin_Manual/*输入电压或输入控制量手动*/ <= ManualAccMin/*手动油门下限*/]
    settings: description=本路径的判据/动作：[Vin_Manual <= ManualAccMin]。执行次序1；条件成立才执行本箭头动作。
  (junction 102) -> (junction 105)
    settings: description=无附加条件的迁移路径，执行次序1；沿本图当前连接推进。
  (junction 96) -> (junction 102) : {Vout/*输出电压或输出控制量*/ =ManualAccMin/*手动油门下限*/;
      |  ServoCtrlFlag/*油泵给定选择标志*/ = PG_ServoCtrlMode_ManualAccMin/*手动油门下限*/;}
    settings: description=本路径的判据/动作：{Vout =ManualAccMin; ServoCtrlFlag = PG_ServoCtrlMode_ManualAccMin;}。执行次序1；条件成立才执行本箭头动作。
  (junction 100) -> (junction 102)
    settings: description=无附加条件的迁移路径，执行次序1；沿本图当前连接推进。
  (junction 93) -> (junction 100) : {Vout/*输出电压或输出控制量*/ =ManualAccMax/*手动油门上限*/;
      |  ServoCtrlFlag/*油泵给定选择标志*/ = PG_ServoCtrlMode_ManualAccMax/*手动油门上限*/;}
    settings: description=本路径的判据/动作：{Vout =ManualAccMax; ServoCtrlFlag = PG_ServoCtrlMode_ManualAccMax;}。执行次序1；条件成立才执行本箭头动作。
  (junction 106) -> (junction 100)
    settings: description=无附加条件的迁移路径，执行次序1；沿本图当前连接推进。
  (junction 3) -> (junction 106) : {Vout/*输出电压或输出控制量*/ =Vin_Start/*输入电压或输入控制量起动*/;
      |  ServoCtrlFlag/*油泵给定选择标志*/ = PG_CtrlMode_Start/*起动*/;}
    settings: description=本路径的判据/动作：{Vout =Vin_Start; ServoCtrlFlag = PG_CtrlMode_Start;}。执行次序1；条件成立才执行本箭头动作。
  data: EngineCtrlMode input uint8; Vin_Origin input single; Vin_Start input single; Vin_Idle input single; CloseLoopMin input single; CloseLoopMax input single; Vin_Stop input single; Vin_Manual input single; ManualAccMin input single; PG_ServoCtrlMode_CloseLoop parameter uint8; PG_ServoCtrlMode_CloseLoopMax parameter uint8; PG_ServoCtrlMode_CloseLoopMin parameter uint8; PG_ServoCtrlMode_ManualAcc parameter uint8; PG_ServoCtrlMode_ManualAccMax parameter uint8; PG_ServoCtrlMode_ManualAccMin parameter uint8; ServoCtrlFlag output uint8 =0; Vout output single =0; ManualAccMax input single; PG_CtrlMode_Start parameter uint8; PG_CtrlMode_ManualAcc parameter uint8; PG_CtrlMode_CloseLoop parameter uint8; PG_CtrlMode_Stop parameter uint8; PG_CtrlMode_Origin parameter uint8

== stateflow chart turbo_controller/SaveData/Hold ==
  note: 产生0～255循环的记录序号
      |
      | 每次执行先判断当前Out是否已达到255：达到就置0，否则加1。序列循环为…253、254、255、0、1…
      | 。
      |
      | 这里先判断再递增，避免uint8在255上继续加1触发溢出诊断。它是记录顺序标记，不是秒数；记录间
      | 隔取决于父级调用频率。一个序号重复出现也不一定表示数据重复，因为每256次调用会正常回到相同
      | 编号。
  (default) -> (junction 26)
    settings: description=无附加条件的迁移路径，执行次序1；沿本图当前连接推进。
  (junction 26) -> (junction 3) [order 1] : [Out/*记录序号*/ >= 255]
    settings: description=本路径的判据/动作：[Out >= 255]。执行次序1；条件成立才执行本箭头动作。
  (junction 26) -> (junction 43) [order 2] : {Out/*输出*/ ++;}
    settings: description=本路径的判据/动作：{Out ++;}。执行次序2；条件成立才执行本箭头动作。
  (junction 3) -> (junction 55) : {Out/*输出*/ = 0;}
    settings: description=本路径的判据/动作：{Out = 0;}。执行次序1；条件成立才执行本箭头动作。
  (junction 55) -> (junction 43)
    settings: description=无附加条件的迁移路径，执行次序1；沿本图当前连接推进。
  (junction 43) -> (junction 71)
    settings: description=无附加条件的迁移路径，执行次序1；沿本图当前连接推进。
  data: Out output uint8 =0

== stateflow chart turbo_controller/CLM/ClpControl/Aim__Parameter_Calculate/Aim_AccMaxMin_Cal1/HoldFirst/Hold ==
  note: 第一次进入时只记住一次反馈转速
      |
      | 输入Nc_First来自父级的当前滤波转速。Flag_First尚未置位时，把这个值保存到Nc_First_Hold；以
      | 后每次执行都输出保存值，不再跟着实时反馈改变。
      |
      | 例如第一次输入40000，后续变到40500、41000，本图输出仍是40000。这样M_Rate_Limiter有稳定的起
      | 点，能够自己向装订目标推进，而不会被实时反馈不断重新拉回。
      |
      | 这个保持只对本次图表生命周期有效；什么时候重新初始化由父级动作子系统和图表配置决定。它不会
      | 暂停模型，也不会要求转速一直保持在40000。
  (default) -> (junction 26)
    settings: description=无附加条件的迁移路径，执行次序1；沿本图当前连接推进。
  (junction 26) -> (junction 3) [order 1] : [true/*真值*/ == Flag_First/*标志首次*/]
    settings: description=本路径的判据/动作：[true == Flag_First]。执行次序1；条件成立才执行本箭头动作。
  (junction 26) -> (junction 43) [order 2] : {Out/*输出*/ = Nc_First/*控制器转速变量首次*/;
      | Nc_First_Hold/*控制器转速变量首次保持*/=Nc_First/*控制器转速变量首次*/;
      | Flag_First/*标志首次*/ = true/*真值*/;}
    settings: description=本路径的判据/动作：{Out = Nc_First; Nc_First_Hold=Nc_First; Flag_First = true;}。执行次序2；条件成立才执行本箭头动作。
  (junction 3) -> (junction 55) : {Out/*输出*/ =Nc_First_Hold/*控制器转速变量首次保持*/;}
    settings: description=本路径的判据/动作：{Out =Nc_First_Hold;}。执行次序1；条件成立才执行本箭头动作。
  (junction 55) -> (junction 43)
    settings: description=无附加条件的迁移路径，执行次序1；沿本图当前连接推进。
  (junction 43) -> (junction 71)
    settings: description=无附加条件的迁移路径，执行次序1；沿本图当前连接推进。
  data: Out output single =0; Flag_First local boolean =0; Nc_First input single =0; Nc_First_Hold local single =0
